simulink model "BlocoHidraulicoLAC_closeLoop"  (R2026a)
settings: Solver=ode15s  StopTime=5  FixedStep=0.001  MaxStep=1e-4
values from neighbouring files (symbols this model uses):
  Gamma = sys_d.B    [sintese_lqi_luenberger_lac.m]    (also in sintese_lqi_luenberger_lac_bateria_de_ensaio.m)
  K_i = -K_aug(3)    [sintese_lqi_luenberger_lac.m]    (also in sintese_lqi_luenberger_lac_bateria_de_ensaio.m)
  K_lqr = [K_pos, K_vel]    [sintese_lqi_luenberger_lac.m]    (also in sintese_lqi_luenberger_lac_bateria_de_ensaio.m)
  L_obs = place(Phi', Cx', polos_obs)'    [sintese_lqi_luenberger_lac.m]    (also in sintese_lqi_luenberger_lac_bateria_de_ensaio.m)
  Phi = sys_d.A    [sintese_lqi_luenberger_lac.m]    (also in sintese_lqi_luenberger_lac_bateria_de_ensaio.m)
undefined symbols (not defined in the file or in its folder): sigbuilder_block
(part 4 of 4)

== matlab function BlocoHidraulicoLAC_closeLoop/ BlocoHidraulicoLAC 2 ==
  settings: updateMethod=DISCRETE
  data: duty_cycle_lac input; u_mcv input; u_pfv input; u_irl input; u_orl input; P_supply output; P_roda output; dt input; x_mm output
function [ P_supply, P_roda, x_mm] = fcn(duty_cycle_lac,u_mcv, u_pfv, u_irl, u_orl,  dt)
%#codegen
% BLOCO DE PLANTA FÍSICA HIDRO-MECÂNICA ATUALIZADO (CINEMÁTICA DO FUSO REAL)
% Inputs:
%   u_mcv, u_pfv, u_irl, u_orl : Sinais ON/OFF (0 ou 1)
%   duty_cycle_lac             : Sinal de comando do LAC (-1.0 a 1.0 ou 0 a 1)
%   dt                         : Passo de amostragem (ex: 0.001)
% Outputs:
%   x_ponto                    : Velocidade instantânea do êmbolo [m/s]
%   P_supply                   : Pressão de suprimento (Nó p1) [Pa]
%   P_roda                     : Pressão na roda (Nó p3) [Pa]
%   x_mm                       : DESLOCAMENTO DO LAC EM MILÍMETROS [mm]

%% 1. PARAMETROS FIXOS DO SISTEMA (Valores validados pelo usuário)
rho     = 850;          % Densidade do fluido [kg/m^3]
beta    = 1.5e9;        % Módulo volumétrico [Pa]
A_lac   = 2.85e-4;      % Área do êmbolo do LAC [m^2]
V10     = 2.0e-5;       % Volume morto inicial [m^3]
%Valor sugerido para teste: Mude de V10 = 2.0e-5 para V10 = 1.0e-5 (\(10\text{ mL}\)).

% % Parâmetro Mecânico Real do Motor/Fuso
% K_drv   = 0.7e-4;      % Ganho real: m/s por unidade de comando (Velocidade máx: 0.269 mm/s)
% tau_m   = 0.020;        % Constante de tempo elétrica/mecânica do motor (ex: 20 ms)

% Parâmetros Reais Extraídos da Bancada (Escala 0-100)
K_drv   = 0.085;    % Média calibrada para a zona útil de controle (10% a 30%)
tau_m   = 0.140;      % Constante de aceleração real do motor (140 ms)

% Válvulas (Orifícios)
Cd      = 0.62;         %1.0;          % Coeficiente de descarga uniforme
A_max   = 3.5e-6;      %8.47e-7;      % Área máxima de passagem das válvulas [m^2]
tau_v   = 0.005;        % Constante de tempo do carretel [s]
pr      = 0.0;          % Pressão do reservatório [Pa]

% Volumes e Compliances dos Nós 2 e 3
C2      = 5.0e-12;      % Compliance da linha principal [m^3/Pa]
% C2      = 2.0e-12;      % REDUZIDO: Linha principal do bloco mais rígida
C3      = 4.5e-12; %2.5e-11;      % Compliance total do caliper [m^3/Pa]
% Valor sugerido para teste: Experimente testar C3 = 1.2e-12 ou C3 = 8.5e-13.


%% 2. INICIALIZAÇÃO DOS ESTADOS INTERNOS (PERSISTENT)
persistent p1 p2 p3 x x_dot a_mcv a_pfv a_irl a_orl

if isempty(p1)
    p1     = 0.0;  p2    = 0.0;  p3    = 0.0;
    x      = 0.0;  x_dot = 0.0;
    a_mcv  = 0.0;  a_pfv = 0.0;  a_irl = 0.0;  a_orl = 0.0;
end

%% 3. DINÂMICA DOS CARRETÉIS DAS VÁLVULAS
a_mcv = a_mcv + (dt / tau_v) * (-a_mcv + double(u_mcv));
a_pfv = a_pfv + (dt / tau_v) * (-a_pfv + double(u_pfv));
a_irl = a_irl + (dt / tau_v) * (-a_irl + double(u_irl));
a_orl = a_orl + (dt / tau_v) * (-a_orl + double(u_orl));

a_mcv = max(0.0, min(1.0, a_mcv));
a_pfv = max(0.0, min(1.0, a_pfv));
a_irl = max(0.0, min(1.0, a_irl));
a_orl = max(0.0, min(1.0, a_orl));

%% 4. CÁLCULO DAS VAZÕES INSTANTÂNEAS
A_eff_mcv = a_mcv * A_max;
A_eff_pfv = a_pfv * A_max;
A_eff_irl = a_irl * A_max; % Acoplamento IRL/ORL conforme lógica
A_eff_orl = a_orl * A_max;

dp_pfv = p1 - p2;
dp_mcv = p2 - pr;
dp_irl = p2 - p3;
dp_orl = p3 - pr;

Q_pfv = Cd * A_eff_pfv * sign(dp_pfv) * sqrt(2 * abs(dp_pfv) / rho);
Q_mcv = Cd * A_eff_mcv * sign(dp_mcv) * sqrt(2 * abs(dp_mcv) / rho);
Q_irl = Cd * A_eff_irl * sign(dp_irl) * sqrt(2 * abs(dp_irl) / rho);
Q_orl = Cd * A_eff_orl * sign(dp_orl) * sqrt(2 * abs(dp_orl) / rho);

%% 5. EQUAÇÕES DIFERENCIAIS DA PLANTA (EDOs)

% --- Mecânica Cinemática Real do Atuador do LAC ---
% Em vez de força, o comando de PWM gera uma velocidade alvo ditada pelo fuso.
% O motor possui um pequeno atraso físico de resposta (atraso de primeira ordem tau_m)
%x_dot_alvo = double(duty_cycle_lac) * K_drv;
x_dot_alvo = (double(duty_cycle_lac) / 100) * K_drv; % Garante que 50 vire 0.5

x_ddot     = (1 / tau_m) * (-x_dot + x_dot_alvo);

% --- Dinâmica Hidráulica ---
V1 = V10 - A_lac * x;
if V1 < 1.0e-7
    V1 = 1.0e-7;
end
p1_dot = (beta / V1) * (A_lac * x_dot - Q_pfv);
p2_dot = (1 / C2) * (Q_pfv - Q_mcv - Q_irl);
p3_dot = (1 / C3) * (Q_irl - Q_orl);

%% 6. INTEGRAÇÃO NUMÉRICA (Método de Euler)
x_dot = x_dot + x_ddot * dt;
x     = x + x_dot * dt;

% [ADICIONE ESTA LINHA AQUI]: Proteção de Fim de Curso Máximo do LAC
if x >= 0.0537
    x = 0.0537;
    x_dot = max(0.0, x_dot); % Impede o pistão de continuar avançando se bater no fundo
end

p1    = p1 + p1_dot * dt;
p2    = p2 + p2_dot * dt;
p3    = p3 + p3_dot * dt;

% Saturações físicas de fim de curso e cavitação
p1 = max(0.0, p1);
p2 = max(0.0, p2);
p3 = max(0.0, p3);
x  = max(0.0, x); % Impede deslocamento negativo na parede inicial

%% 7. ATRIBUIÇÃO DAS SAÍDAS DO BLOCO
%x_ponto  = x_dot;
P_supply = p1/6894.757;
P_roda   = p3/6894.757;
x_mm     = x * 1000; % Converte de metros [m] para milímetros [mm] para leitura real

end



% esse codigo funcionou parcialmente
% function [P_supply, P_roda, x_ponto] = fcn(duty_cycle_lac, u_mcv, u_pfv, u_irl, u_orl,  dt)
% %#codegen
% % BLOCO DE PLANTA FÍSICA HIDRO-MECÂNICA (LAC + VALVULAS + CALIPER)
% % Inputs vindos da ECU:
% %   u_mcv, u_pfv, u_irl, u_orl : Sinais ON/OFF (0 ou 1)
% %   duty_cycle_lac             : Sinal PWM do motor do LAC (0.0 a 1.0)
% %   dt                         : Passo de amostragem da simulação (ex: 0.001)
% % Outputs para os sensores:
% %   x_ponto                    : Velocidade do êmbolo do LAC [m/s]
% %   P_supply                   : Pressão de suprimento (Nó p1 do LAC) [Pa]
% %   P_roda                     : Pressão na roda/caliper (Nó p3) [Pa]
% 
% %% 1. PARAMETROS FIXOS DO SISTEMA (Altere conforme seu projeto)
% % Fluido e Geometria do LAC
% rho     = 850;          % Densidade do fluido [kg/m^3]
% beta    = 1.5e9;        % Módulo volumétrico [Pa]
% A_lac   = 2.85e-4;       % Área do êmbolo do LAC [m^2]
% V10     = 2.0e-5;       % Volume morto inicial [m^3]
% 
% % Mecânica do Atuador do LAC
% m_lac   = 1.5;          % Massa equivalente do êmbolo/motor [kg]
% b_lac   = 2000;          % Coeficiente de amortecimento [N*s/m]
% k_lac   = 0.0;          % Rigidez de retorno mecânico [N/m]
% K_motor = 0.538;          % Ganho de força do motor por Duty Cycle [N]
% V_max   = 24;           % Tensão de alimentação nominal [V]
% 
% % Válvulas (Orifícios)
% Cd      = 1.0;         % Coeficiente de descarga uniforme
% A_max   = 8.47e-7;      % Área máxima de passagem das válvulas [m^2]
% tau_v   = 0.005;        % Constante de tempo do carretel [s]
% pr      = 0.0;          % Pressão do reservatório [Pa]
% 
% % Volumes e Compliances dos Nós 2 e 3
% C2      = 5.0e-12;      % Compliance da linha principal [m^3/Pa]
% C3      = 2.5e-11;      % Compliance total do caliper (Fluido + Pastilha) [m^3/Pa]
% 
% %% 2. INICIALIZAÇÃO DOS ESTADOS INTERNOS (PERSISTENT)
% persistent p1 p2 p3 x x_dot a_mcv a_pfv a_irl a_orl
% 
% if isempty(p1)
%     p1     = 0.0;  p2    = 0.0;  p3    = 0.0;
%     x      = 0.0;  x_dot = 0.0;
%     a_mcv  = 0.0;  a_pfv = 0.0;  a_irl = 0.0;  a_orl = 0.0;
% end
% 
% %% 3. DINÂMICA DOS CARRETÉIS DAS VÁLVULAS (Filtros de comando)
% a_mcv = a_mcv + (dt / tau_v) * (-a_mcv + double(u_mcv));
% a_pfv = a_pfv + (dt / tau_v) * (-a_pfv + double(u_pfv));
% a_irl = a_irl + (dt / tau_v) * (-a_irl + double(u_irl));
% a_orl = a_orl + (dt / tau_v) * (-a_orl + double(u_orl));
% 
% % Garantir limites físicos das aberturas [0, 1]
% a_mcv = max(0.0, min(1.0, a_mcv));
% a_pfv = max(0.0, min(1.0, a_pfv));
% a_irl = max(0.0, min(1.0, a_irl));
% a_orl = max(0.0, min(1.0, a_orl));
% 
% %% 4. CÁLCULO DAS VAZÕES INSTANTÂNEAS (Modelo de Orifício)
% % Áreas instantâneas
% A_eff_mcv = a_mcv * A_max;
% A_eff_pfv = a_pfv * A_max;
% A_eff_irl = a_irl * A_max;
% A_eff_orl = a_orl * A_max;
% 
% % Diferenciais de pressão
% dp_pfv = p1 - p2;
% dp_mcv = p2 - pr;
% dp_irl = p2 - p3;
% dp_orl = p3 - pr;
% 
% % Equação de escoamento não-linear
% Q_pfv = Cd * A_eff_pfv * sign(dp_pfv) * sqrt(2 * abs(dp_pfv) / rho);
% Q_mcv = Cd * A_eff_mcv * sign(dp_mcv) * sqrt(2 * abs(dp_mcv) / rho);
% Q_irl = Cd * A_eff_irl * sign(dp_irl) * sqrt(2 * abs(dp_irl) / rho);
% Q_orl = Cd * A_eff_orl * sign(dp_orl) * sqrt(2 * abs(dp_orl) / rho);
% 
% %% 5. EQUAÇÕES DIFERENCIAIS DA PLANTA (EDOs)
% 
% % --- Dinâmica Mecânica do LAC ---
% % Força elétrica gerada pelo PWM (Limitada entre 0 e K_motor)
% F_motor = double(max(0.0, min(1.0, duty_cycle_lac))) * K_motor;
% % Força de reação hidráulica contrária que o fluido faz no êmbolo
% F_hidr  = A_lac * p1; 
% 
% % Aceleração do LAC (x_ponto_ponto)
% x_ddot = (1 / m_lac) * (F_motor - b_lac * x_dot - k_lac * x - F_hidr);
% 
% % --- Dinâmica Hidráulica (Pressões) ---
% % Nó 1: Volume variável do LAC
% V1 = V10 - A_lac * x;
% if V1 < 1.0e-7 % Proteção contra fim de curso/divisão por zero
%     V1 = 1.0e-7;
% end
% p1_dot = (beta / V1) * (A_lac * x_dot - Q_pfv);
% 
% % Nó 2: Linha principal
% p2_dot = (1 / C2) * (Q_pfv - Q_mcv - Q_irl);
% 
% % Nó 3: Caliper da Roda
% p3_dot = (1 / C3) * (Q_irl - Q_orl);
% 
% %% 6. INTEGRAÇÃO NUMÉRICA (Método de Euler)
% x_dot = x_dot + x_ddot * dt;
% x     = x + x_dot * dt;
% p1    = p1 + p1_dot * dt;
% p2    = p2 + p2_dot * dt;
% p3    = p3 + p3_dot * dt;
% 
% % Saturações de segurança física (Pressão não pode ser negativa -> Cavitação)
% p1 = max(0.0, p1);
% p2 = max(0.0, p2);
% p3 = max(0.0, p3);
% x  = max(0.0, x); % Êmbolo não volta além da posição de repouso
% 
% %% 7. ATRIBUIÇÃO DAS SAÍDAS DO BLOCO
% x_ponto  = x_dot;
% P_supply = p1/6894.757;
% P_roda   = p3/6894.757;
% 
% end










% function [Pw_psi, Ps_psi, x_mm] = MKc2_step(PWM, MCV, PFV, IRL, ORL)
% %#codegen
% % Planta hidráulica de freio (AEB/ACC) simplificada: LAC + válvulas + caliper
% % Entradas:
% %   PWM ∈ [0..100] ou [0..1]  (comando do LAC)
% %   MCV, PFV, IRL, ORL ∈ {0,1} (1=acionada)
% % Convenção:
% %   MCV=1 isola do reservatório (sem alívio); MCV=0 abre LAC→reservatório
% %   PFV=1 abre LAC→linha; IRL=1 abre linha→caliper; ORL=1 abre caliper→reservatório
% % Saídas:
% %   Pw_psi (psi) — pressão na roda/caliper
% %   Ps_psi (psi) — pressão de suprimento (câmara do LAC)
% %   x_mm   (mm)  — deslocamento do LAC
% 
% % ---------------------------------
% % ESTADOS
% % ---------------------------------
% persistent x Ps Pw Vgap a_line a_orl a_mcv
% if isempty(x)
%     x     = 0.0;    % m
%     Ps    = 0.0;    % Pa
%     Pw    = 0.0;    % Pa
%     Vgap  = 6.3e-6; % m^3 (≈ 6.3 mL) — folga inicial da roda (ajuste)
%     a_line= 0.0;    % m^2 área efetiva S↔W (PFV∧IRL)
%     a_orl = 0.0;    % m^2 área efetiva W→R (ORL)
%     a_mcv = 0.0;    % m^2 área efetiva S→R (MCV aberta)
% end
% 
% % ---------------------------------
% % PARÂMETROS (ajuste para o hardware)
% % ---------------------------------
% % Discretização
% Ts = 1e-3;                  % s
% 
% % LAC (cinemática aberta, sem PI interno)
% A_p   = 2.85e-4;            % m^2 (área efetiva do pistão)
% x_max = 0.0537;             % m  (curso máx)
% x_ds  = 0.0050;             % m  (dead stroke visto no LAC)
% K_drv_mps_per_pct = 2.69e-4;% m/s por %PWM (caracterizado no real)
% F_max = 2500.0;             % N  (força máx no êmbolo a 100% PWM) — ajuste
% use_droop = true;           % queda de velocidade com pressão (v→0 quando A_p*Ps→F_max)
% 
% % Fluido / compressibilidade efetiva
% rho     = 1050.0;           % kg/m^3
% betaS0  = 1.0e9;            % Pa    (suprimento)
% betaW0  = 1.0e9;            % Pa    (roda)
% k_betaS = 0.0e-9;           % 1/Pa  (enrijecimento com P) — ajuste fino
% k_betaW = 2.0e-9;           % 1/Pa  (enrijecimento com P) — ajuste fino
% Vs0     = 4.0e-6;           % m^3   (volume efetivo suprimento)
% Vw0     = 11.3e-6;          % m^3   (volume efetivo roda/linha, sem folga)
% 
% % Orifícios equivalentes (Cd*A) em ON (65 cm^3/s @ 25 bar → ~9.4e-7 m^2)
% CdA_LINE_ON = 9.4e-7;       % m^2 (S↔W quando PFV∧IRL abertos)
% CdA_ORL_ON  = 9.4e-7;       % m^2 (W→R quando ORL aberta)
% CdA_MCV_ON  = 9.4e-7;       % m^2 (S→R quando MCV aberta)
% 
% % Fugas (opcionais)
% CdA_leak_S  = 0.0e-9;       % m^2 (S→R)
% CdA_leak_W  = 0.0e-9;       % m^2 (W→R)
% 
% % Dinâmica eletromecânica das válvulas (1ª ordem)
% tau_val = 0.02;             % s (10–30 ms típico)
% 
% % Conversão
% PA_PER_PSI = 6894.757;
% 
% % ---------------------------------
% % ENTRADAS E FLAGS
% % ---------------------------------
% % PWM como %
% if PWM <= 1.0
%     pwm_pct = 100.0*max(0.0,min(1.0,PWM));
% else
%     pwm_pct = max(0.0,min(100.0,PWM));
% end
% 
% MCV_isol = (MCV ~= 0);  % 1=isola
% PFV_open = (PFV ~= 0);  % 1=aberta
% IRL_open = (IRL ~= 0);  % 1=aberta
% ORL_open = (ORL ~= 0);  % 1=aberta
% 
% % ---------------------------------
% % LAC — deslocamento a partir do PWM (com droop de carga)
% % ---------------------------------
% P_port = Ps;           % pressão na face do êmbolo (≈Ps se MCV=1; ≈0 se MCV=0)
% if ~MCV_isol
%     P_port = 0.0;
% end
% 
% v_nom = K_drv_mps_per_pct * pwm_pct;   % m/s
% if use_droop
%     droop = max(0.0, 1.0 - (A_p*P_port)/max(F_max,1.0));
% else
%     droop = 1.0;
% end
% v = v_nom * droop;                     % m/s
% 
% % integrar x com saturação
% x = x + Ts*v;
% if x < 0.0,    x = 0.0;    end
% if x > x_max,  x = x_max;  end
% 
% % Vazão do pistão (só após dead stroke)
% if x <= x_ds
%     Qp = 0.0;
% else
%     Qp = A_p * v;   % m^3/s
% end
% 
% % ---------------------------------
% % Válvulas — áreas efetivas com atraso (1ª ordem)
% % ---------------------------------
% line_cmd = CdA_LINE_ON * double(PFV_open && IRL_open);
% orl_cmd  = CdA_ORL_ON  * double(ORL_open);
% mcv_cmd  = CdA_MCV_ON  * double(~MCV_isol);
% 
% a_line = a_line + Ts*(line_cmd - a_line)/max(tau_val,Ts);
% a_orl  = a_orl  + Ts*(orl_cmd  - a_orl )/max(tau_val,Ts);
% a_mcv  = a_mcv  + Ts*(mcv_cmd  - a_mcv )/max(tau_val,Ts);
% 
% % ---------------------------------
% % Lei de orifício — vazões assinadas
% % ---------------------------------
% % Enquanto houver folga (Vgap>0), a pressão na roda é ~0.
% Pw_for_line = Pw;
% if Vgap > 0.0
%     Pw_for_line = 0.0;
% end
% 
% Q_sw   = orifice_signed(Ps, Pw_for_line, a_line, rho);  % S↔W
% Q_wr   = orifice_signed(Pw, 0.0,       a_orl,  rho);    % W→R
% Q_sr   = orifice_signed(Ps, 0.0,       a_mcv,  rho);    % S→R
% Q_lk_S = orifice_signed(Ps, 0.0,       CdA_leak_S, rho);
% Q_lk_W = orifice_signed(Pw, 0.0,       CdA_leak_W, rho);
% 
% % ---------------------------------
% % Dead stroke como volume de folga (consome Q_sw até zerar Vgap)
% % ---------------------------------
% if (Vgap > 0.0) && (Q_sw > 0.0) && (a_line > 0.0)
%     Vgap = Vgap - Ts*Q_sw;
%     if Vgap < 0.0, Vgap = 0.0; end
% end
% 
% % ---------------------------------
% % Balanço de compressibilidade
% % ---------------------------------
% betaS = betaS0 * (1.0 + k_betaS*Ps);
% betaW = betaW0 * (1.0 + k_betaW*Pw);
% 
% % Suprimento (sempre integra)
% Ps_dot = (betaS / max(Vs0,eps)) * ( Qp - Q_sr - Q_sw - Q_lk_S );
% Ps = Ps + Ts*Ps_dot;
% if Ps < 0.0, Ps = 0.0; end
% 
% % Roda: só integra após fechar folga; antes, mantém Pw≈0
% if Vgap > 0.0
%     Pw = 0.0;
% else
%     Pw_dot = (betaW / max(Vw0,eps)) * ( Q_sw - Q_wr - Q_lk_W );
%     Pw = Pw + Ts*Pw_dot;
%     if Pw < 0.0, Pw = 0.0; end
% end
% 
% % ---------------------------------
% % SAÍDAS
% % ---------------------------------
% Pw_psi = Pw / PA_PER_PSI;
% Ps_psi = Ps / PA_PER_PSI;
% x_mm   = x  * 1e3;
% 
% end
% 
% % -------- orifício com sinal (local) --------
% function q = orifice_signed(Pu, Pd, CdA, rho)
% %#codegen
% if CdA <= 0.0
%     q = 0.0;
%     return;
% end
% dP = Pu - Pd;
% if dP > 0.0
%     q = CdA * sqrt(2.0 * dP / rho);
% elseif dP < 0.0
%     q = -CdA * sqrt(2.0 * (-dP) / rho);
% else
%     q = 0.0;
% end
% end
% % function [Pw_psi, Ps_psi, x_mm] = MKc2_step(PWM, MCV, PFV, IRL, ORL)
% % %#codegen
% % % Planta hidráulica MKc2 (LAC + válvulas) sem controle, com lei de orifício.
% % % Entradas (escalares):
% % %   PWM ∈ [0..100] (%) ou [0..1]       – comando do motor do LAC (abrevia: velocidade)
% % %   MCV, PFV, IRL, ORL ∈ {0,1}         – válvulas ON/OFF (1=acionada)
% % % Convenção das válvulas (compatível com o prompt):
% % %   MCV: 1=isola reservatório (câmara do LAC fechada); 0=alívio LAC→reservatório
% % %   PFV: 1=abre LAC→linha
% % %   IRL: 1=abre linha→caliper (convenção pedida: 1=ABERTA)
% % %   ORL: 1=abre caliper→reservatório
% % % Saídas:
% % %   Pw_psi – pressão no caliper (psi)
% % %   Ps_psi – pressão de suprimento/câmara do LAC (psi)
% % %   x_mm   – deslocamento do LAC (mm)
% % 
% % % ==========================
% % % ESTADOS (persistentes)
% % % ==========================
% % persistent x Ps Pw
% % if isempty(x)
% %     x  = 0.0;   % m  (posição do LAC)
% %     Ps = 0.0;   % Pa (pressão na câmara do LAC / suprimento)
% %     Pw = 0.0;   % Pa (pressão na roda/caliper)
% % end
% % 
% % % ==========================
% % % PARÂMETROS (ajustáveis)
% % % ==========================
% % % Discretização
% % Ts = 1e-3;                  % s (use igual ao passo do modelo)
% % 
% % % LAC (geometria e curso)
% % A_p   = 2.85e-4;            % m^2  (área efetiva do pistão do LAC)
% % x_max = 0.0537;             % m    (curso máximo ~53,7 mm)
% % x_ds  = 0.0050;             % m    (dead stroke ~5,0 mm – sem geração de pressão)
% % 
% % % LAC (cinemática aberta – sem PI dentro do bloco)
% % % K_drv dado em m/s por %PWM (valores coletados do sistema)
% % K_drv_mps_per_pct = 2.69e-4;   % m/s por %PWM
% % 
% % % Fluido / compressibilidade efetiva (ajuste pela validação)
% % rho   = 1050.0;             % kg/m^3
% % betaS = 1.0e9;              % Pa (módulo efetivo nó S – LAC)
% % betaW = 1.0e9;              % Pa (módulo efetivo nó W – roda)
% % Vs0   = 4.0e-6;             % m^3 (volume efetivo no nó S – ordem de mL)
% % Vw0   = 11.3e-6;            % m^3 (volume efetivo no nó W – ~ V_line_dead + V_dead_max)
% % 
% % % Orifícios equivalentes (Cd*A) quando ABERTOS (valores a partir de 65 cm^3/s @ 25 bar)
% % % CdA ≈ Q_nom / sqrt(2*ΔP/ρ) → ≈ 9.4e-7 m^2 (ajuste fino em bancada/simulação)
% % CdA_LINE_ON = 9.4e-7;       % m^2 (PFV & IRL ABERTAS: LAC ↔ caliper)
% % CdA_ORL_ON  = 9.4e-7;       % m^2 (ORL ABERTA: caliper → reservatório)
% % CdA_MCV_ON  = 9.4e-7;       % m^2 (MCV ABERTA: LAC → reservatório)
% % 
% % % Fugas pequenas (opcionais; ajudam estabilidade numérica)
% % CdA_leak_S  = 0.0e-9;       % m^2 (fuga S→reservatório)
% % CdA_leak_W  = 0.0e-9;       % m^2 (fuga W→reservatório)
% % 
% % % Conversão
% % PA_PER_PSI = 6894.757;      % Pa/psi
% % 
% % % ==========================
% % % PROCESSAMENTO DE ENTRADAS
% % % ==========================
% % % Normalização de PWM (aceita % ou [0..1])
% % if PWM > 1.0
% %     pwm_pct = PWM;           % já está em %
% % else
% %     pwm_pct = 100.0*PWM;     % converte fração → %
% % end
% % if pwm_pct < 0.0;   pwm_pct = 0.0;   end
% % if pwm_pct > 100.0; pwm_pct = 100.0; end
% % 
% % % Flags de válvula (1=ON)
% % MCV_isol = (MCV ~= 0);   % 1=isola (fechada p/ reservatório)
% % PFV_open = (PFV ~= 0);   % 1=aberta
% % IRL_open = (IRL ~= 0);   % 1=aberta (convenção pedida)
% % ORL_open = (ORL ~= 0);   % 1=aberta
% % 
% % % ==========================
% % % CINEMÁTICA DO LAC (sem PI)
% % % ==========================
% % % Fonte de velocidade: v = K_drv * (%PWM)
% % v_cmd = K_drv_mps_per_pct * pwm_pct;   % m/s (sempre positiva neste modelo)
% % 
% % % Integração de posição com saturação mecânica
% % x = x + Ts * v_cmd;
% % if x < 0.0
% %     x = 0.0;
% % end
% % if x > x_max
% %     x = x_max;
% % end
% % 
% % % Vazão volumétrica do pistão (só após dead stroke)
% % if x <= x_ds
% %     Qp = 0.0;            % m^3/s – tomando folgas; sem geração de pressão
% % else
% %     Qp = A_p * v_cmd;    % m^3/s – fluxo injetado no nó S
% % end
% % 
% % % ==========================
% % % HIDRÁULICA – LEI DE ORIFÍCIO
% % % ==========================
% % % Áreas ativas conforme comandos
% % CdA_line = 0.0;
% % if PFV_open && IRL_open
% %     CdA_line = CdA_LINE_ON;      % LAC ↔ roda
% % end
% % 
% % CdA_orl = 0.0;
% % if ORL_open
% %     CdA_orl = CdA_ORL_ON;        % roda → reservatório
% % end
% % 
% % CdA_mcv = 0.0;
% % if ~MCV_isol
% %     CdA_mcv = CdA_MCV_ON;        % LAC → reservatório
% % end
% % 
% % % Vazões assinadas (sentido positivo do primeiro nó para o segundo)
% % % Nodos: S (Ps), W (Pw), R (Pr≈0)
% % Pr  = 0.0;
% % Q_sw = orifice_signed(Ps, Pw, CdA_line, rho);   % S→W
% % Q_wr = orifice_signed(Pw, Pr,  CdA_orl,  rho);  % W→R
% % Q_sr = orifice_signed(Ps, Pr,  CdA_mcv,  rho);  % S→R
% % 
% % % Fugas (sempre para reservatório)
% % Q_leak_S = orifice_signed(Ps, Pr, CdA_leak_S, rho);
% % Q_leak_W = orifice_signed(Pw, Pr, CdA_leak_W, rho);
% % 
% % % Balanço de massa/compressibilidade
% % % dP/dt = (β/V) * (ΣQ_entrada − ΣQ_saída)
% % Ps_dot = (betaS / Vs0) * ( Qp - Q_sr - Q_sw - Q_leak_S );
% % Pw_dot = (betaW / Vw0) * ( Q_sw - Q_wr - Q_leak_W );
% % 
% % % Integração de pressões
% % Ps = Ps + Ts * Ps_dot;
% % Pw = Pw + Ts * Pw_dot;
% % 
% % % Limites físicos
% % if Ps < 0.0; Ps = 0.0; end
% % if Pw < 0.0; Pw = 0.0; end
% % 
% % % ==========================
% % % SAÍDAS
% % % ==========================
% % Pw_psi = Pw / PA_PER_PSI;
% % Ps_psi = Ps / PA_PER_PSI;
% % x_mm   = x  * 1e3;
% % 
% % 
% % 
% % 
% % 
% % 
% % 
% % 
% % 
% % 
% % 
% % 
% % 
% % 
% % 
% % 
% % 
% % 
% % 
% % 
% % 
% % Ps_dot = (Ps_beta_s/Vs) * ( Qp - Q_sr - sum_i * Q_swi - Q_leak_S );
% % Pwi_dot = (Pwi_beta_w_i/Vw_i) * ( Q_swi - Q_wri - Q_leak_Wi );
% % 
% % 
% % end
% % 
% % % ==========================
% % % Função local: lei de orifício com sinal
% % % q > 0 quando Pu>Pd (escoa de Pu→Pd); q < 0 quando Pu<Pd.
% % % ==========================
% % function q = orifice_signed(Pu, Pd, CdA, rho)
% % %#codegen
% % if CdA <= 0.0
% %     q = 0.0;
% %     return;
% % end
% % dP = Pu - Pd;
% % if dP > 0.0
% %     q = CdA * sqrt(2.0 * dP / rho);
% % elseif dP < 0.0
% %     q = -CdA * sqrt(2.0 * (-dP) / rho);
% % else
% %     q = 0.0;
% % end
% % end
% % 
% % % function [Pw_psi, Ps_psi, x_mm] = MKc2_step(PWM, MCV, PFV, IRL, ORL)
% % % %#codegen
% % % % MKc2_step — planta hidráulica (LAC + válvulas) com lei de orifício, pronta p/ portabilidade
% % % % Entradas (escalares):
% % % %   PWM ∈ [0..100] (%) ou [0..1]   — comando do motor/atuador do LAC
% % % %   MCV, PFV, IRL, ORL ∈ {0,1}     — comandos ON/OFF das válvulas
% % % % Saídas:
% % % %   Pw_psi — pressão no caliper (psi)
% % % %   Ps_psi — pressão na câmara do LAC (psi)
% % % %   x_mm   — deslocamento do LAC (mm)
% % % 
% % % % ESTADOS
% % % persistent x v Ps Pw
% % % if isempty(x)
% % %     x  = 0.0;   % m
% % %     v  = 0.0;   % m/s
% % %     Ps = 0.0;   % Pa
% % %     Pw = 0.0;   % Pa
% % % end
% % % 
% % % % ==========================
% % % % PARÂMETROS AJUSTÁVEIS
% % % % ==========================
% % % % Discretização
% % % Ts = 1e-3;        % s (use o mesmo passo do modelo)
% % % 
% % % % Mecânica do LAC
% % % x_max = 0.043;    % m (curso máximo 43 mm)
% % % x_ds  = 0.005;    % m (dead stroke 5 mm)
% % % M_eq  = 0.50;     % kg (massa/inerção equivalente)
% % % B_m   = 20.0;     % N*s/m (atrito viscoso)
% % % K_f   = 200.0;    % N (força efetiva do atuador a PWM=1)
% % % A_p   = 1.0e-4;   % m^2 (área efetiva do êmbolo ~ diâmetro ≈ 11.3 mm)
% % % 
% % % % Hidráulica (compressibilidade e volumes efetivos)
% % % beta_s = 1.5e9;   % Pa (módulo volumétrico efetivo da câmara do LAC)
% % % beta_w = 1.5e9;   % Pa (módulo volumétrico efetivo do caliper/linha roda)
% % % Vs0    = 4.0e-6;  % m^3 (volume efetivo câmara LAC ~ 4 mL)
% % % Vw0    = 12.0e-6; % m^3 (volume efetivo caliper/linha ~ 12 mL)
% % % rho    = 1050.0;  % kg/m^3 (densidade do fluido)
% % % Pr     = 0.0;     % Pa (reservatório em pressão de referência ≈ 0 gauge)
% % % 
% % % % Áreas efetivas de orifício (Cd*A) quando ABERTAS (ON):
% % % CdA_LINE_ON = 1.0e-7;  % m^2 (linha LAC↔caliper, PFV e IRL ABERTAS)
% % % CdA_ORL_ON  = 1.2e-7;  % m^2 (retorno caliper→reservatório, ORL ABERTA)
% % % CdA_MCV_ON  = 1.0e-7;  % m^2 (alívio LAC→reservatório, MCV ABERTA)
% % % 
% % % % Pequenas fugas opcionais (mantêm numérica estável quando tudo fechado)
% % % CdA_leak_S  = 0.0e-9;  % m^2 (fuga câmara LAC→reservatório)
% % % CdA_leak_W  = 0.0e-9;  % m^2 (fuga caliper→reservatório)
% % % 
% % % % Conversão
% % % PA_PER_PSI = 6894.757; % Pa/psi
% % % 
% % % % ==========================
% % % % CONVENÇÃO DE COMANDO (PORTABILIDADE)
% % % % 1 = acionado (ON), 0 = desacionado (OFF)
% % % % - MCV=1: isola do reservatório (sem alívio). MCV=0: alívio LAC→reservatório.
% % % % - PFV=1: abre LAC→linha.
% % % % - IRL=1: ABRE para o caliper (convenção pedida). IRL=0: isola caliper.
% % % % - ORL=1: abre retorno caliper→reservatório.
% % % % ==========================
% % % MCV_isol  = (MCV ~= 0);   % MCV=1 isola; MCV=0 alivia
% % % PFV_open  = (PFV ~= 0);   % PFV=1 abre
% % % IRL_open  = (IRL ~= 0);   % IRL=1 abre (conforme solicitado)
% % % ORL_open  = (ORL ~= 0);   % ORL=1 abre
% % % 
% % % % Normalização PWM
% % % if PWM > 1.0
% % %     PWM = PWM/100.0;
% % % end
% % % if PWM < 0.0; PWM = 0.0; end
% % % if PWM > 1.0; PWM = 1.0; end
% % % 
% % % % ==========================
% % % % MECÂNICA DO LAC
% % % % ==========================
% % % % Reação hidráulica no êmbolo (porto da câmara do LAC)
% % % P_port = Ps;
% % % 
% % % % Forças e aceleração
% % % F_m = K_f * PWM;              % N (atuador)
% % % F_h = A_p * P_port;           % N (reação do fluido)
% % % a   = (F_m - B_m*v - F_h)/M_eq;
% % % 
% % % % Integração com saturações de curso
% % % v = v + Ts*a;
% % % x = x + Ts*v;
% % % 
% % % if x < 0.0
% % %     x = 0.0;
% % %     if v < 0.0; v = 0.0; end
% % % end
% % % if x > x_max
% % %     x = x_max;
% % %     if v > 0.0; v = 0.0; end
% % % end
% % % 
% % % % Vazão do êmbolo (só conta após dead stroke)
% % % if x <= x_ds
% % %     Qp = 0.0;      % m^3/s (tomada de folgas; não gera pressão)
% % % else
% % %     Qp = A_p * v;  % m^3/s (assinada: positiva comprime, negativa suga)
% % % end
% % % 
% % % % ==========================
% % % % HIDRÁULICA COM LEI DE ORIFÍCIO
% % % % ==========================
% % % % Áreas ativas conforme comandos
% % % CdA_line = 0.0;
% % % if PFV_open && IRL_open
% % %     CdA_line = CdA_LINE_ON;
% % % end
% % % 
% % % CdA_orl = 0.0;
% % % if ORL_open
% % %     CdA_orl = CdA_ORL_ON;
% % % end
% % % 
% % % CdA_mcv = 0.0;
% % % if ~MCV_isol
% % %     % MCV aberta ao reservatório ⇒ alívio LAC→reservatório
% % %     CdA_mcv = CdA_MCV_ON;
% % % end
% % % 
% % % % Vazões (assinadas pelo gradiente de pressão)
% % % Q_sw = orifice_signed(Ps, Pw, CdA_line, rho);      % S→W (positivo se Ps>Pw)
% % % Q_wr = orifice_signed(Pw, Pr,  CdA_orl,  rho);     % W→R (positivo se Pw>Pr)
% % % Q_sr = orifice_signed(Ps, Pr,  CdA_mcv,  rho);     % S→R (positivo se Ps>Pr)
% % % 
% % % % Fugas opcionais (sempre para reservatório)
% % % Q_leak_S = orifice_signed(Ps, Pr, CdA_leak_S, rho);
% % % Q_leak_W = orifice_signed(Pw, Pr, CdA_leak_W, rho);
% % % 
% % % % Balanços de volume (compressibilidade)
% % % Ps_dot = (beta_s / Vs0) * ( Qp - Q_sr - Q_sw - Q_leak_S );
% % % Pw_dot = (beta_w / Vw0) * ( Q_sw - Q_wr - Q_leak_W );
% % % 
% % % % Integração de pressões
% % % Ps = Ps + Ts * Ps_dot;
% % % Pw = Pw + Ts * Pw_dot;
% % % 
% % % % Saturações físicas
% % % if Ps < 0.0; Ps = 0.0; end
% % % if Pw < 0.0; Pw = 0.0; end
% % % 
% % % % ==========================
% % % % SAÍDAS
% % % % ==========================
% % % Pw_psi = Pw / PA_PER_PSI;
% % % Ps_psi = Ps / PA_PER_PSI;
% % % x_mm   = x * 1e3;
% % % 
% % % end
% % % 
% % % % ==========================
% % % % Função local: lei de orifício com sinal
% % % %   Retorna vazão positiva no sentido Pu→Pd quando Pu>Pd,
% % % %   e negativa quando Pu<Pd.
% % % % ==========================
% % % function q = orifice_signed(Pu, Pd, CdA, rho)
% % % %#codegen
% % % if CdA <= 0
% % %     q = 0.0;
% % %     return;
% % % end
% % % dP = Pu - Pd;
% % % if dP > 0
% % %     q = CdA * sqrt(2.0 * dP / rho);
% % % elseif dP < 0
% % %     q = -CdA * sqrt(2.0 * (-dP) / rho);
% % % else
% % %     q = 0.0;
% % % end
% % % end
% % % % function [Ps_psi, Pw_psi, x_mm] = MKc2_step(PWM, MCV, PFV, IRL, ORL) 
% % % % % MKc2_step — modelo simplificado (teórico) do módulo hidráulico com LAC e válvulas. 
% % % % % Entradas: 
% % % % % PWM [0..100] (%) ou [0..1], MCV/PFV/IRL/ORL ∈ {0,1} 
% % % % % Saídas: 
% % % % % Pw_psi — pressão no caliper (psi) 
% % % % % Ps_psi — pressão na câmara do LAC (psi) 
% % % % % x_mm — deslocamento do LAC (mm)
% % % % 
% % % % % Estados persistentes 
% % % % persistent x v Ps Pw 
% % % % if isempty(x) 
% % % % 	x = 0.0; % m 
% % % % 	v = 0.0; % m/s 
% % % % 	Ps = 0.0; % Pa 
% % % % 	Pw = 0.0; % Pa 
% % % % end
% % % % 
% % % % % Constantes e parâmetros (ajuste conforme necessário) 
% % % % Ts = 1e-3; % s (usar igual ao sample time do bloco) 
% % % % x_max = 0.043; % m (43 mm) 
% % % % x_ds = 0.005; % m (5 mm dead stroke) 
% % % % M_eq = 0.50; % kg 
% % % % B_m = 20.0; % N*s/m 
% % % % K_f = 200.0; % N (força efetiva max. do atuador no êmbolo) 
% % % % A_p = 1.0e-4; % m^2 (área efetiva do êmbolo) 
% % % % Pmax = 10.3e6; % Pa (~1500 psi) 
% % % % k_p = 250.0; % 1/m (≈0.25 por mm) 
% % % % tau_h = 5e-3; % s (dinâmica hidráulica do LAC) 
% % % % tau_mcv = 3e-3; % s (alívio via MCV) 
% % % % tau_line= 2e-3; % s (equalização LAC↔caliper) 
% % % % tau_orl = 8e-3; % s (alívio via ORL) 
% % % % tau_leak= 0.5; % s (retenção/fuga lenta) 
% % % % PA_PER_PSI = 6894.757; % Pa por psi
% % % % 
% % % % % Normalização PWM para [0,1] 
% % % % if PWM > 1.0 
% % % % 	PWM = PWM/100.0; 
% % % % end 
% % % % if PWM < 0.0 
% % % % 	PWM = 0.0; 
% % % % end 
% % % % if PWM > 1.0 
% % % % 	PWM = 1.0; 	
% % % % end
% % % % 
% % % % % 1) Força do atuador e pressão no porto do LAC (para reação hidráulica) 
% % % % % Assumimos lógica de válvulas: 
% % % % % MCV=1 fecha reservatório (isola); MCV=0 abre (alívio). 
% % % % % PFV=1 abre LAC→linha; IRL=0 abre linha→caliper; ORL=1 alívio caliper→reservatório. 
% % % % % Pressão que reage no êmbolo: 
% % % % if MCV==0 
% % % %     P_port = 0.0; % câmara conectada ao reservatório 
% % % % else % MCV=1: câmara pode estar isolada (PFV=0) ou conectada à linha (PFV=1) 
% % % %     if PFV==1 && IRL==0 && ORL==0 % LAC conectado ao caliper (sem alívio) 
% % % %     % aproximamos reação no êmbolo pela pressão do LAC (Ps), 
% % % %     % que tenderá a equalizar com Pw (feito mais abaixo) 
% % % %         P_port = Ps; 
% % % %     elseif PFV==0 % LAC isolado da linha, câmara fechada 
% % % %         P_port = Ps; 
% % % %     else % Outras combinações (ex.: IRL=1 ou ORL=1) → pouca reação efetiva no êmbolo
% % % %         P_port = Ps; 
% % % %     end 
% % % % end
% % % % 
% % % % F_m = K_f * PWM; % N 
% % % % F_h = A_p * P_port; % N (oposição hidráulica) 
% % % % a = (F_m - B_m*v - F_h)/M_eq; % m/s^2
% % % % 
% % % % % Integração mecânica 
% % % % v = v + Ts*a; 
% % % % x = x + Ts*v;
% % % % 
% % % % % Limites mecânicos (batente e não recuar abaixo de 0) 
% % % % if x < 0.0 
% % % %     x = 0.0; 
% % % % 	if v < 0.0; v = 0.0; 
% % % % 	end 
% % % % end 
% % % % if x > x_max 
% % % %     x = x_max; 
% % % % 	if v > 0.0; v = 0.0; 
% % % % 	end 
% % % % end
% % % % 
% % % % % 2) Pressão alvo no LAC por dead stroke + exponencial 
% % % % if x <= x_ds 
% % % % 	Pstat = 0.0; 
% % % % else 
% % % % 	Pstat = Pmax * (1.0 - exp(-k_p * (x - x_ds))); 
% % % % end
% % % % 
% % % % % 3) Dinâmica da pressão na câmara do LAC (Ps) 
% % % % if MCV==1 % Isolado do reservatório → Ps tende a Pstat 
% % % % 	Ps = Ps + Ts*(Pstat - Ps)/tau_h; 
% % % % else % Aberto ao reservatório → Ps tende a 0 
% % % % 	Ps = Ps + Ts*(0.0 - Ps)/tau_mcv; 
% % % % end 
% % % % if Ps < 0.0 
% % % % 	Ps = 0.0; 
% % % % end
% % % % 
% % % % % 4) Dinâmica da pressão no caliper (Pw) 
% % % % if ORL==1 % Alívio direto ao reservatório domina 
% % % % 	Pw = Pw + Ts*(0.0 - Pw)/tau_orl; 
% % % % else % Sem alívio 
% % % % 	if (IRL==0) && (PFV==1) && (MCV==1) % Linha LAC↔caliper conectada e LAC isolado do reservatório 
% % % % 		Pw = Pw + Ts*(Ps - Pw)/tau_line; 
% % % % 	else % Isolado/retido (IRL=1 ou PFV=0 ou MCV=0) → retenção com fuga lenta 
% % % % 		Pw = Pw + Ts*(0.0 - Pw)/tau_leak; 
% % % % 	end 
% % % % end 
% % % % if Pw < 0.0 
% % % % 	Pw = 0.0; 
% % % % end
% % % % 
% % % % % 5) Saídas convertidas 
% % % % Pw_psi = Pw / PA_PER_PSI; 
% % % % Ps_psi = Ps / PA_PER_PSI; 
% % % % x_mm = x * 1e3;
% % % % 
% % % % end
% % % % % function [P_sup, P_wh4, x_dot] = BlocoHidraulicoLAC_FisicaRigorosa(PWM_LAC, CMD_MCV, CMD_PFV, CMD_IRL, CMD_ORL)
% % % % %     % #####################################################################
% % % % %     % MODELO HIDRÁULICO EAB REFINADO - COMPORTAMENTO NÃO-LINEAR (PSI)
% % % % %     % #####################################################################
% % % % % 
% % % % %     % --- PARÂMETROS CONSTANTES ---
% % % % %     dt = 0.001;                 % Passo de tempo (1 ms)
% % % % %     P_atm = 101325;             % Pressão atm (Pa)
% % % % %     P_max_pa = 190 * 1e5;       % Limite físico do sistema: 190 bar em Pascal
% % % % % 
% % % % %     % Parâmetros Geométricos do LAC
% % % % %     A_p = 2.85e-4;              % Área efetiva do pistão do LAC (m²)
% % % % %     K_drv = 2.69e-4;            % m/s por %PWM
% % % % %     x_max = 0.0537;             % Curso máximo do LAC (53.7 mm)
% % % % % 
% % % % %     % Parâmetros do Caliper 4 e Linha
% % % % %     D_caliper = 0.040;          % Diâmetro do pistão da pinça (40 mm)
% % % % %     A_caliper = pi*(D_caliper/2)^2; 
% % % % %     deadstroke_max = 0.005;     % Folga pastilha-disco (5 mm)
% % % % %     V_dead_max = A_caliper * deadstroke_max; % Volume do deadstroke (~6.28 mL)
% % % % %     V_line_dead = 5e-6;         % Volume morto da linha rígida isolada (5 mL)
% % % % % 
% % % % %     % Parâmetros de Restrição da Válvula Solenoide (65 cm³/s @ 25 bar)
% % % % %     Q_nom = 65e-6;              
% % % % %     dP_nom = 25e5;              
% % % % %     C_v = Q_nom / sqrt(dP_nom); 
% % % % % 
% % % % %     % --- VARIÁVEIS DE ESTADO (PERSISTENT) ---
% % % % %     persistent x_lac P_sup_state P_wh4_state V_to_caliper
% % % % %     if isempty(x_lac)
% % % % %         x_lac = 0.0;            % Posição inicial do LAC (m)
% % % % %         P_sup_state = P_atm;     % Pressão inicial de suprimento (Pa)
% % % % %         P_wh4_state = P_atm;     % Pressão inicial na roda (Pa)
% % % % %         V_to_caliper = 0.0;     % Volume acumulado enviado para a pinça (m³)
% % % % %     end
% % % % % 
% % % % %     % --- 1. DINÂMICA DE DESLOCAMENTO DO LAC (FIM DE CURSO RIGOROSO) ---
% % % % %     x_dot = 0.0;
% % % % %     if x_lac < x_max
% % % % %         x_dot = PWM_LAC * K_drv;
% % % % %         x_lac = x_lac + x_dot * dt;
% % % % %         if x_lac > x_max
% % % % %             x_lac = x_max;
% % % % %             x_dot = 0.0; % Parou no batente mecânico
% % % % %         end
% % % % %     end
% % % % %     Q_lac = A_p * x_dot; % Vazão volumétrica gerada pelo movimento
% % % % % 
% % % % %     % --- 2. LÓGICA DIGITAL DAS VÁLVULAS ---
% % % % %     open_MCV = (CMD_MCV == 0);
% % % % %     open_PFV = (CMD_PFV == 1);
% % % % %     open_IRL = (CMD_IRL == 0);
% % % % %     open_ORL = (CMD_ORL == 1);
% % % % % 
% % % % %     % --- 3. EQUAÇÕES DE ESCOAMENTO (BERNOULLI COM ACOPLAMENTO) ---
% % % % %     Q_irl = 0;
% % % % %     if open_IRL
% % % % %         dP_irl = P_sup_state - P_wh4_state;
% % % % %         Q_irl = C_v * sign(dP_irl) * sqrt(abs(dP_irl));
% % % % %     end
% % % % % 
% % % % %     Q_orl = 0;
% % % % %     if open_ORL
% % % % %         dP_orl = P_wh4_state - P_atm;
% % % % %         Q_orl = C_v * sign(dP_orl) * sqrt(abs(dP_orl));
% % % % %     end
% % % % % 
% % % % %     % --- 4. COMPRESSIBILIDADE E COMPLACÊNCIA NÃO-LINEAR (EFEITO EXPONENCIAL) ---
% % % % %     % Módulo de elasticidade dinâmico do fluido (varia com a pressão para simular rigidez)
% % % % %     Beta_fluid = 1.4e9; 
% % % % % 
% % % % %     % Dinâmica da Pressão de Suprimento (P_sup)
% % % % %     % NOTA: Se a IRL fechar, V_line_dead é minúsculo, fazendo a pressão disparar rápido!
% % % % %     dP_sup_dt = (Beta_fluid / V_line_dead) * (Q_lac - Q_irl);
% % % % %     P_sup_state = P_sup_state + dP_sup_dt * dt;
% % % % % 
% % % % %     % Dinâmica da Pressão de Roda (P_wh4) com Deadstroke e Rigidez de Pastilha
% % % % %     Q_net_wheel = Q_irl - Q_orl;
% % % % %     V_to_caliper = max(0, V_to_caliper + Q_net_wheel * dt);
% % % % % 
% % % % %     if V_to_caliper <= V_dead_max
% % % % %         % FASE 1: Consumindo os 5mm de Deadstroke. Pressão manométrica é ZERO.
% % % % %         P_wh4_state = P_atm;
% % % % %     else
% % % % %         % FASE 2: Contato com o disco. O volume excedente esmaga a mola não-linear da pastilha.
% % % % %         V_compressed = V_to_caliper - V_dead_max;
% % % % % 
% % % % %         % Função exponencial de rigidez: a pressão ganha curvatura com o esmagamento volumétrico
% % % % %         % Adota uma aproximação clássica de complacência de freios (p = k * V^1.5 ou exponencial)
% % % % %         P_gauge = 0.5e5 * (V_compressed / 1e-7)^1.8; 
% % % % %         P_wh4_state = P_atm + P_gauge;
% % % % %     end
% % % % % 
% % % % %     % --- 5. SATURAÇÃO FÍSICA E LIMITE DE 190 BAR ---
% % % % %     if P_sup_state > P_max_pa, P_sup_state = P_max_pa; end
% % % % %     if P_wh4_state > P_max_pa, P_wh4_state = P_max_pa; end
% % % % %     if P_sup_state < P_atm, P_sup_state = P_atm; end
% % % % %     if P_wh4_state < P_atm, P_wh4_state = P_atm; end
% % % % % 
% % % % %     % --- 6. CONVERSÃO FINAL DAS SAÍDAS PARA PSI ---
% % % % %     % 1 Pascal = 0.0001450377377 PSI
% % % % %     pa_to_psi = 1.450377e-4;
% % % % %     P_sup = (P_sup_state - P_atm) * pa_to_psi;
% % % % %     P_wh4 = (P_wh4_state - P_atm) * pa_to_psi;
% % % % % end
% % % % % % function [P_sup, P_wh4, x_dot] = hydraulic_block_EAB(PWM_LAC, CMD_MCV, CMD_PFV, CMD_IRL, CMD_ORL)
% % % % % %     % #####################################################################
% % % % % %     % MODELO DO BLOCO HIDRÁULICO EAB - CALIPER 4 (CAMINHO VERDE E AZUL)
% % % % % %     % Inputs:
% % % % % %     %   PWM_LAC : Sinal de comando do atuador linear (0 a 100%)
% % % % % %     %   CMD_MCV : Comando da Válvula de Controle do Cilindro Mestre (0=NO, 1=Fechada)
% % % % % %     %   CMD_PFV : Comando da Válvula de Alimentação do LAC (0=NC, 1=Aberta)
% % % % % %     %   CMD_IRL : Comando da Válvula de Entrada da Roda (0=NO, 1=Fechada)
% % % % % %     %   CMD_ORL : Comando da Válvula de Saída da Roda (0=NC, 1=Aberta)
% % % % % %     % #####################################################################
% % % % % % 
% % % % % %     % --- PARÂMETROS CONSTANTES DO SISTEMA ---
% % % % % %     dt = 0.001;                 % Passo de tempo da simulação (1 ms)
% % % % % %     Beta = 1.4e9;               % Bulk Modulus do fluido de freio (Pa)
% % % % % %     P_atm = 101325;             % Pressão atmosférica/reservatório (Pa)
% % % % % %     rho = 900;                  % Densidade do fluido de freio (kg/m³)
% % % % % % 
% % % % % %     % Parâmetros do LAC
% % % % % %     A_p = 2.85e-4;              % Área efetiva do pistão do LAC (m²)
% % % % % %     K_drv = 2.69e-4;            % Ganho de velocidade do pistão (m/s por %PWM)
% % % % % % 
% % % % % %     % Parâmetros do Caliper 4
% % % % % %     D_caliper = 0.040;          % ASSUMIDO: Diâmetro do pistão da pinça (40 mm = 0.04 m)
% % % % % %     A_caliper = pi*(D_caliper/2)^2; % Área do pistão da pinça (m²)
% % % % % %     deadstroke_max = 0.005;     % Folga pastilha-disco (5 mm = 0.005 m)
% % % % % %     V_dead_max = A_caliper * deadstroke_max; % Volume morto máximo (m³)
% % % % % %     V_line = 10e-6;             % ASSUMIDO: Volume da linha hidráulica (10 mL)
% % % % % % 
% % % % % %     % Parâmetros das Válvulas (Nominal: 65 cm³/s @ 25 bar)
% % % % % %     Q_nom = 65e-6;              % Vazão nominal (m³/s)
% % % % % %     dP_nom = 25e5;              % Diferença de pressão nominal (Pa)
% % % % % %     C_v = Q_nom / sqrt(dP_nom); % Coeficiente de restrição calculado
% % % % % % 
% % % % % %     % --- VARIÁVEIS DE ESTADO (PERSISTENT) ---
% % % % % %     persistent P_sup_state P_wh4_state V_dead_consumed
% % % % % %     if isempty(P_sup_state)
% % % % % %         P_sup_state = P_atm;     % Pressão inicial de suprimento (Pascal)
% % % % % %         P_wh4_state = P_atm;     % Pressão inicial na roda (Pascal)
% % % % % %         V_dead_consumed = 0.0;   % Volume consumido no deslocamento da pastilha
% % % % % %     end
% % % % % % 
% % % % % %     % --- 1. DINÂMICA DO ATUADOR LAC ---
% % % % % %     % Velocidade e vazão volumétrica gerada pelo LAC
% % % % % %     x_dot = PWM_LAC * K_drv;
% % % % % %     Q_lac = A_p * x_dot;
% % % % % % 
% % % % % %     % --- 2. LÓGICA DIGITAL DAS VÁLVULAS (NO / NC) ---
% % % % % %     % MCV (Normalmente Aberta)
% % % % % %     if CMD_MCV == 0, open_MCV = 1; else, open_MCV = 0; end
% % % % % %     % PFV (Normalmente Fechada)
% % % % % %     if CMD_PFV == 1, open_PFV = 1; else, open_PFV = 0; end
% % % % % %     % IRL (Normalmente Aberta)
% % % % % %     if CMD_IRL == 0, open_IRL = 1; else, open_IRL = 0; end
% % % % % %     % ORL (Normalmente Fechada)
% % % % % %     if CMD_ORL == 1, open_ORL = 1; else, open_ORL = 0; end
% % % % % % 
% % % % % %     % --- 3. CÁLCULO DAS VAZÕES ENTRE CÂMARAS ---
% % % % % %     % Vazão pela PFV (Suprimento LAC -> Nó Central do Caminho Verde)
% % % % % %     % Se fechada, a vazão é zero. Se aberta, depende do gradiente de pressão.
% % % % % %     Q_pfv = 0;
% % % % % %     if open_PFV == 1
% % % % % %         dP_pfv = P_sup_state - P_atm; % Alimentação vinda do reservatório/acumulador
% % % % % %         Q_pfv = C_v * sign(dP_pfv) * sqrt(abs(dP_pfv));
% % % % % %     end
% % % % % % 
% % % % % %     % Vazão de Entrada na Roda 4 via IRL (Caminho Verde -> Caliper 4)
% % % % % %     Q_irl = 0;
% % % % % %     if open_IRL == 1
% % % % % %         dP_irl = P_sup_state - P_wh4_state;
% % % % % %         Q_irl = C_v * sign(dP_irl) * sqrt(abs(dP_irl));
% % % % % %     end
% % % % % % 
% % % % % %     % Vazão de Saída da Roda 4 via ORL (Caliper 4 -> Linha de Retorno Azul)
% % % % % %     Q_orl = 0;
% % % % % %     if open_ORL == 1
% % % % % %         dP_orl = P_wh4_state - P_atm; % Retorno direto para o reservatório (Caminho Azul)
% % % % % %         Q_orl = C_v * sign(dP_orl) * sqrt(abs(dP_orl));
% % % % % %     end
% % % % % % 
% % % % % %     % --- 4. BALANÇO DE PRESSÃO E CONSUMO DE DEADSTROKE ---
% % % % % % 
% % % % % %     % Atualização da Pressão de Suprimento (Nó do LAC)
% % % % % %     % O acúmulo de pressão depende do escoamento gerado e do que sai pelas válvulas
% % % % % %     dP_sup_dt = (Beta / V_line) * (Q_lac - Q_irl);
% % % % % %     P_sup_state = P_sup_state + dP_sup_dt * dt;
% % % % % %     if P_sup_state < P_atm, P_sup_state = P_atm; end % Saturação física
% % % % % % 
% % % % % %     % Dinâmica da Roda 4 (Caliper) incorporando o Deadstroke
% % % % % %     Q_net_wheel = Q_irl - Q_orl;
% % % % % % 
% % % % % %     if V_dead_consumed < V_dead_max && Q_net_wheel > 0
% % % % % %         % Fase de aproximação: Consome o volume morto, pressão não sobe significativamente
% % % % % %         V_dead_consumed = V_dead_consumed + Q_net_wheel * dt;
% % % % % %         dP_wh4_dt = 0; 
% % % % % %         P_wh4_state = P_atm; % Mantém em pressão manométrica zero
% % % % % %     elseif V_dead_consumed >= V_dead_max
% % % % % %         % Fase de contato: Pastilha encostou no disco, pressão sobe rigidamente
% % % % % %         dP_wh4_dt = (Beta / V_line) * Q_net_wheel;
% % % % % %         P_wh4_state = P_wh4_state + dP_wh4_dt * dt;
% % % % % %     else
% % % % % %         % Caso haja alívio de pressão e retorno da pastilha
% % % % % %         if P_wh4_state > P_atm
% % % % % %             dP_wh4_dt = (Beta / V_line) * Q_net_wheel;
% % % % % %             P_wh4_state = P_wh4_state + dP_wh4_dt * dt;
% % % % % %         else
% % % % % %             P_wh4_state = P_atm;
% % % % % %             V_dead_consumed = max(0, V_dead_consumed + Q_net_wheel * dt);
% % % % % %             dP_wh4_dt = 0;
% % % % % %         end
% % % % % %     end
% % % % % % 
% % % % % %     % Saturação inferior de segurança física
% % % % % %     if P_wh4_state < P_atm, P_wh4_state = P_atm; end
% % % % % % 
% % % % % %     % --- 5. CONVERSÃO PARA UNIDADE COMUM (PSI) ---
% % % % % %     P_sup = (P_sup_state - P_atm) / 1.45038e-4;
% % % % % %     P_wh4 = (P_wh4_state - P_atm) / 1.45038e-4;
% % % % % % end
% % % % % % 
% % % % % % % function [Psup_dot, Pw_dot, x_dot, Qlac, Qmcv, Qin, Qout] = BlocoHidraulicoLAC( ...
% % % % % % %     u_pwm, mcv_open, pfv_open, irl_open, orl_open, Psup, Pw, x)
% % % % % % % % Modelo hidráulico MK C2 (EAB/ACC) — nó de suprimento (Psup) e roda/caliper (Pw)
% % % % % % % % Convenção: 1 = válvula ABERTA (mcv_open, pfv_open, irl_open, orl_open)
% % % % % % % % Saídas: derivadas Psup_dot, Pw_dot, x_dot e vazões Qlac, Qmcv, Qin, Qout
% % % % % % % % Unidades internas: SI (Pa, m, m^3/s, kg/m^3). Pressões são ABSOLUTAS.
% % % % % % % 
% % % % % % % % ===== Fluido / referências =====
% % % % % % % rho    = 850;           % kg/m^3 (DOT típico)
% % % % % % % P_atm  = 1.01325e5;     % Pa
% % % % % % % Pret   = P_atm;         % reservatório (referência)
% % % % % % % DP_MIN = 500;           % Pa — faixa morta para ΔP ~ 0 (evita ruído numérico)
% % % % % % % 
% % % % % % % % ===== Geometria LAC (MK C2) =====
% % % % % % % D_mc   = 19.05e-3;                  % m (êmbolo master)
% % % % % % % A_p    = pi*(D_mc/2)^2;             % m^2 (~2.85e-4)
% % % % % % % V_t    = 15.3e-6;                   % m^3 (15.3 mL) volume deslocável
% % % % % % % x_max  = V_t / A_p;                 % m (~0.0537 m)
% % % % % % % 
% % % % % % % % ===== Driver do fuso (MK C2) =====
% % % % % % % mm_per_rev = 42.63/73;              % mm/rev
% % % % % % % m_per_rev  = mm_per_rev * 1e-3;     % m/rev
% % % % % % % f_max_hz   = 46;                    % rev/s
% % % % % % % K_drv      = (f_max_hz * m_per_rev) / 100;  % (m/s)/%PWM
% % % % % % % 
% % % % % % % % ===== Volumes efetivos (ajustáveis por aplicação) =====
% % % % % % % V0_sup = 6.0e-5;      % m^3 (manifold/suprimento ~ 60 mL)
% % % % % % % Vw     = 1.0e-5;      % m^3 (linha+caliper roda ~ 10 mL)
% % % % % % % V_min  = 1.0e-6;      % m^3 (proteção numérica)
% % % % % % % 
% % % % % % % % ===== Chaves de modelo =====
% % % % % % % USE_BETA_VAR = true;    % true: β(P) variável (ar+fluido); false: β constante
% % % % % % % USE_VVAR     = true;    % true: Vsup(x) = V0_sup − A_p*x; false: Vsup constante
% % % % % % % 
% % % % % % % % ===== β constante (validação) =====
% % % % % % % beta_const = 0.08e9;    % Pa (≈80 MPa efetivo)
% % % % % % % 
% % % % % % % % ===== β(P) variável (realismo com ar) =====
% % % % % % % beta_liq = 1.5e9;       % Pa (fluido puro)
% % % % % % % eps0     = 0.03;        % fração volumétrica de ar a 1 atm (2–6% típico)
% % % % % % % gamma_ar = 1.4;         % razão de calores específicos do ar
% % % % % % % 
% % % % % % % % ===== Válvulas (lei do orifício) =====
% % % % % % % Cv   = 0.62;            % coeficiente de descarga
% % % % % % % Amcv = 3.0e-6;          % m^2 (MCV)
% % % % % % % Airl = 3.0e-7;          % m^2 (IRL)
% % % % % % % Aorl = 3.0e-7;          % m^2 (ORL)
% % % % % % % 
% % % % % % % % ===== Vazamentos opcionais (fechamento de balanço) =====
% % % % % % % K_leak_sup = 0.0;       % m^3/(s·Pa) — vazamento Psup→reservatório (default 0)
% % % % % % % K_leak_w   = 0.0;       % m^3/(s·Pa) — vazamento Pw→reservatório (default 0)
% % % % % % % 
% % % % % % % % ===== Sanitização das entradas =====
% % % % % % % u_pwm    = max(min(u_pwm, 100), -100);
% % % % % % % mcv_open = double(mcv_open ~= 0);
% % % % % % % pfv_open = double(pfv_open ~= 0);
% % % % % % % irl_open = double(irl_open ~= 0);
% % % % % % % orl_open = double(orl_open ~= 0);
% % % % % % % Psup     = max(Psup, Pret);   % absolutas ≥ pressão do reservatório
% % % % % % % Pw       = max(Pw,   Pret);
% % % % % % % x        = min(max(x, 0), x_max);
% % % % % % % 
% % % % % % % % ===== Cinemática do êmbolo (saturada no curso) =====
% % % % % % % v_cmd = K_drv * u_pwm;               % m/s
% % % % % % % if (x <= 0 && v_cmd < 0)
% % % % % % %     x_dot = 0;
% % % % % % % elseif (x >= x_max && v_cmd > 0)
% % % % % % %     x_dot = 0;
% % % % % % % else
% % % % % % %     x_dot = v_cmd;
% % % % % % % end
% % % % % % % 
% % % % % % % % ===== Vazão do LAC (PFV como chave) =====
% % % % % % % Qlac = pfv_open * A_p * x_dot;       % m^3/s
% % % % % % % 
% % % % % % % % ===== Orifícios com proteção numérica (faixa morta ΔP) =====
% % % % % % % % MCV: Psup ↔ Pret
% % % % % % % dP_mcv = Psup - Pret;
% % % % % % % if abs(dP_mcv) < DP_MIN
% % % % % % %     Qmcv = 0;
% % % % % % % else
% % % % % % %     Qmcv = mcv_open * Cv * Amcv * sign(dP_mcv) * sqrt(2 * abs(dP_mcv) / rho);
% % % % % % % end
% % % % % % % 
% % % % % % % % IRL: Psup ↔ Pw
% % % % % % % dP_irl = Psup - Pw;
% % % % % % % if abs(dP_irl) < DP_MIN
% % % % % % %     Qin = 0;
% % % % % % % else
% % % % % % %     Qin = irl_open * Cv * Airl * sign(dP_irl) * sqrt(2 * abs(dP_irl) / rho);
% % % % % % % end
% % % % % % % 
% % % % % % % % ORL: Pw ↔ Pret
% % % % % % % dP_orl = Pw - Pret;
% % % % % % % if abs(dP_orl) < DP_MIN
% % % % % % %     Qout = 0;
% % % % % % % else
% % % % % % %     Qout = orl_open * Cv * Aorl * sign(dP_orl) * sqrt(2 * abs(dP_orl) / rho);
% % % % % % % end
% % % % % % % 
% % % % % % % % Vazamentos (lineares em ΔP para simplicidade)
% % % % % % % Qleak_sup = K_leak_sup * max(Psup - Pret, 0);   % Psup → reservatório
% % % % % % % Qleak_w   = K_leak_w   * max(Pw   - Pret, 0);   % Pw   → reservatório
% % % % % % % 
% % % % % % % % ===== Volumes (variável no suprimento) =====
% % % % % % % if USE_VVAR
% % % % % % %     Vsup = max(V0_sup - A_p * x, V_min);
% % % % % % % else
% % % % % % %     Vsup = V0_sup;
% % % % % % % end
% % % % % % % 
% % % % % % % % ===== Compressibilidade efetiva =====
% % % % % % % if USE_BETA_VAR
% % % % % % %     % Pressões absolutas para o modelo de ar
% % % % % % %     P_sup_abs = max(Psup, P_atm + 1);
% % % % % % %     P_w_abs   = max(Pw,   P_atm + 1);
% % % % % % % 
% % % % % % %     % fração de ar à pressão atual
% % % % % % %     eps_sup = eps0 * (P_atm / P_sup_abs)^(1 / gamma_ar);
% % % % % % %     eps_w   = eps0 * (P_atm / P_w_abs  )^(1 / gamma_ar);
% % % % % % % 
% % % % % % %     % bulk modulus efetivo
% % % % % % %     beta_sup = 1.0 / (1.0 / beta_liq + eps_sup / (gamma_ar * P_sup_abs));
% % % % % % %     beta_w   = 1.0 / (1.0 / beta_liq + eps_w   / (gamma_ar * P_w_abs));
% % % % % % % else
% % % % % % %     beta_sup = beta_const;
% % % % % % %     beta_w   = beta_const;
% % % % % % % end
% % % % % % % 
% % % % % % % % ===== Dinâmica das pressões =====
% % % % % % % % Balanços de vazão:
% % % % % % % %  Suprimento: entra Qlac; sai Qmcv, Qin, vazamento Qleak_sup
% % % % % % % %  Roda:       entra Qin;  sai Qout, vazamento Qleak_w
% % % % % % % Psup_dot = (beta_sup / Vsup) * (Qlac - Qmcv - Qin - Qleak_sup);
% % % % % % % Pw_dot   = (beta_w   / Vw  ) * (Qin  - Qout - Qleak_w);
% % % % % % % 
% % % % % % % end
% % % % % % % % function [Psup_dot, Pw_dot, x_dot, Qlac, Qmcv, Qin, Qout] = BlocoHidraulicoLAC(u_pwm, mcv_open, pfv_open, irl_open, orl_open, Psup, Pw, x)
% % % % % % % % % Modelo hidráulico LAC – 1=valvula aberta (mcv_open, pfv_open, irl_open, orl_open)
% % % % % % % % % Saídas: derivadas Psup_dot, Pw_dot, x_dot e vazões Qlac, Qmcv, Qin, Qout
% % % % % % % % 
% % % % % % % % % ----- Parâmetros do fluido -----
% % % % % % % % rho   = 850;           % kg/m^3
% % % % % % % % P_atm = 1.01325e5;     % Pa
% % % % % % % % Pret  = P_atm;
% % % % % % % % 
% % % % % % % % % ----- Geometria do LAC -----
% % % % % % % % D_mc  = 19.05e-3;                    % m
% % % % % % % % A_p   = pi*(D_mc/2)^2;               % m^2
% % % % % % % % V_t   = 15.3e-6;                     % m^3
% % % % % % % % x_max = V_t / A_p;                   % m
% % % % % % % % 
% % % % % % % % % ----- Driver do fuso -----
% % % % % % % % mm_per_rev = 42.63/73;               % mm/rev
% % % % % % % % m_per_rev  = mm_per_rev * 1e-3;      % m/rev
% % % % % % % % f_max_hz   = 46;                     % Hz
% % % % % % % % K_drv      = f_max_hz * m_per_rev / 100;  % (m/s)/%PWM
% % % % % % % % 
% % % % % % % % % ----- Volumes -----
% % % % % % % % V0_sup = 6.0e-5;      % m^3 (manifold/suprimento)
% % % % % % % % Vw     = 1.0e-5;      % m^3 (roda/caliper)
% % % % % % % % V_min  = 1.0e-6;      % m^3 (limite numérico)
% % % % % % % % 
% % % % % % % % % ----- Chaves de modelo -----
% % % % % % % % USE_BETA_VAR = true;  % true = beta(P) variável; false = beta constante
% % % % % % % % USE_VVAR     = true;  % true = Vsup(x) variável; false = Vsup constante
% % % % % % % % 
% % % % % % % % % ----- beta constante (validação) -----
% % % % % % % % beta_const = 0.08e9;  % Pa
% % % % % % % % 
% % % % % % % % % ----- beta(P) variável (realismo) -----
% % % % % % % % beta_liq = 1.5e9;     % Pa
% % % % % % % % eps0     = 0.03;      % fração de ar a 1 atm (ajuste)
% % % % % % % % gamma_ar = 1.4;
% % % % % % % % 
% % % % % % % % % ----- Válvulas -----
% % % % % % % % Cv   = 0.62;
% % % % % % % % Amcv = 3.0e-6;        % m^2
% % % % % % % % Airl = 3.0e-7;        % m^2
% % % % % % % % Aorl = 3.0e-7;        % m^2
% % % % % % % % 
% % % % % % % % % ----- Sanitização -----
% % % % % % % % u_pwm    = max(min(u_pwm,100),-100);
% % % % % % % % mcv_open = double(mcv_open ~= 0);
% % % % % % % % pfv_open = double(pfv_open ~= 0);
% % % % % % % % irl_open = double(irl_open ~= 0);
% % % % % % % % orl_open = double(orl_open ~= 0);
% % % % % % % % Psup     = max(Psup, Pret);
% % % % % % % % Pw       = max(Pw,   Pret);
% % % % % % % % x        = min(max(x, 0), x_max);
% % % % % % % % 
% % % % % % % % % ----- Cinemática do pistão -----
% % % % % % % % v_cmd = K_drv * u_pwm;
% % % % % % % % if (x <= 0 && v_cmd < 0)
% % % % % % % %     x_dot = 0;
% % % % % % % % elseif (x >= x_max && v_cmd > 0)
% % % % % % % %     x_dot = 0;
% % % % % % % % else
% % % % % % % %     x_dot = v_cmd;
% % % % % % % % end
% % % % % % % % 
% % % % % % % % % ----- Vazões -----
% % % % % % % % Qlac = pfv_open * A_p * x_dot;
% % % % % % % % 
% % % % % % % % dP_mcv = Psup - Pret;
% % % % % % % % Qmcv   = mcv_open * Cv * Amcv * sign(dP_mcv) * sqrt(2 * abs(dP_mcv) / rho);
% % % % % % % % 
% % % % % % % % dP_irl = Psup - Pw;
% % % % % % % % Qin    = irl_open * Cv * Airl * sign(dP_irl) * sqrt(2 * abs(dP_irl) / rho);
% % % % % % % % 
% % % % % % % % dP_orl = Pw - Pret;
% % % % % % % % Qout   = orl_open * Cv * Aorl * sign(dP_orl) * sqrt(2 * abs(dP_orl) / rho);
% % % % % % % % 
% % % % % % % % % ----- Volumes -----
% % % % % % % % if USE_VVAR
% % % % % % % %     Vsup = max(V0_sup - A_p * x, V_min);
% % % % % % % % else
% % % % % % % %     Vsup = V0_sup;
% % % % % % % % end
% % % % % % % % 
% % % % % % % % % ----- beta efetivo -----
% % % % % % % % if USE_BETA_VAR
% % % % % % % %     P_sup_abs = max(Psup, P_atm + 1);
% % % % % % % %     P_w_abs   = max(Pw,   P_atm + 1);
% % % % % % % %     eps_sup   = eps0 * (P_atm / P_sup_abs)^(1 / gamma_ar);
% % % % % % % %     eps_w     = eps0 * (P_atm / P_w_abs  )^(1 / gamma_ar);
% % % % % % % %     beta_sup  = 1 / (1 / beta_liq + eps_sup / (gamma_ar * P_sup_abs));
% % % % % % % %     beta_w    = 1 / (1 / beta_liq + eps_w   / (gamma_ar * P_w_abs));
% % % % % % % % else
% % % % % % % %     beta_sup  = beta_const;
% % % % % % % %     beta_w    = beta_const;
% % % % % % % % end
% % % % % % % % 
% % % % % % % % % ----- Dinâmica das pressões -----
% % % % % % % % Psup_dot = (beta_sup / Vsup) * (Qlac - Qmcv - Qin);
% % % % % % % % Pw_dot   = (beta_w   / Vw  ) * (Qin  - Qout);
% % % % % % % % end
% % % % % % % % 
% % % % % % % % % function [Psup_dot, Pw_dot, x_dot, Qlac, Qmcv, Qin, Qout] = BlocoHidraulicoLAC( ...
% % % % % % % % %     u_pwm, mcv, pfv, irl, orl, Psup, Pw, x)
% % % % % % % % % % ---------------------------------------------------------------
% % % % % % % % % % Modelo hidráulico LAC — β(P) variável + volume variável
% % % % % % % % % % ---------------------------------------------------------------
% % % % % % % % % 
% % % % % % % % % % ========== FLUIDO ==========
% % % % % % % % % beta_liq = 1.5e9;      % Pa — bulk modulus do fluido puro (sem ar)
% % % % % % % % % eps0     = 0.03;        % fração de ar a P_atm (3% — ajustar ao sistema)
% % % % % % % % % gamma_ar = 1.4;         % razão de calores específicos do ar
% % % % % % % % % P_atm    = 1.01325e5;   % Pa
% % % % % % % % % rho      = 850;         % kg/m³
% % % % % % % % % Pret     = P_atm;       % pressão do reservatório
% % % % % % % % % 
% % % % % % % % % % ========== GEOMETRIA DO LAC ==========
% % % % % % % % % D_mc  = 19.05e-3;
% % % % % % % % % A_p   = pi * (D_mc/2)^2;
% % % % % % % % % V_t   = 15.3e-6;
% % % % % % % % % x_max = V_t / A_p;
% % % % % % % % % 
% % % % % % % % % % ========== DRIVER DO FUSO ==========
% % % % % % % % % mm_per_rev = 42.63 / 73;
% % % % % % % % % m_per_rev  = mm_per_rev * 1e-3;
% % % % % % % % % f_max_hz   = 46;
% % % % % % % % % K_drv      = f_max_hz * m_per_rev / 100;
% % % % % % % % % 
% % % % % % % % % % ========== VOLUMES DE CONTROLE ==========
% % % % % % % % % V0_sup = 6.0e-5;
% % % % % % % % % V0_w   = 1.0e-5;
% % % % % % % % % V_min  = 1.0e-6;
% % % % % % % % % 
% % % % % % % % % Vsup = max(V0_sup - A_p * x, V_min);
% % % % % % % % % Vw   = V0_w;
% % % % % % % % % 
% % % % % % % % % % ========== β EFETIVO = f(P) ==========
% % % % % % % % % %
% % % % % % % % % %  À medida que P sobe, o ar comprime, β cresce, dP/dt acelera
% % % % % % % % % %  ISSO gera a curva exponencial
% % % % % % % % % %
% % % % % % % % % P_sup_abs = max(Psup, P_atm + 1);   % evita divisão por ~0
% % % % % % % % % P_w_abs   = max(Pw,   P_atm + 1);
% % % % % % % % % 
% % % % % % % % % % Fração de ar à pressão atual
% % % % % % % % % eps_sup = eps0 * (P_atm / P_sup_abs)^(1/gamma_ar);
% % % % % % % % % eps_w   = eps0 * (P_atm / P_w_abs  )^(1/gamma_ar);
% % % % % % % % % 
% % % % % % % % % % Bulk modulus efetivo
% % % % % % % % % beta_sup = 1.0 / (1.0/beta_liq + eps_sup/(gamma_ar * P_sup_abs));
% % % % % % % % % beta_w   = 1.0 / (1.0/beta_liq + eps_w  /(gamma_ar * P_w_abs));
% % % % % % % % % 
% % % % % % % % % % ========== VÁLVULAS ==========
% % % % % % % % % Cv   = 0.62;
% % % % % % % % % Amcv = 3.0e-6;
% % % % % % % % % Airl = 3.0e-7;
% % % % % % % % % Aorl = 3.0e-7;
% % % % % % % % % 
% % % % % % % % % % ========== SANITIZAÇÃO ==========
% % % % % % % % % u_pwm = max(min(u_pwm, 100), -100);
% % % % % % % % % mcv   = double(mcv ~= 0);
% % % % % % % % % pfv   = double(pfv ~= 0);
% % % % % % % % % irl   = double(irl ~= 0);
% % % % % % % % % orl   = double(orl ~= 0);
% % % % % % % % % Psup  = max(Psup, Pret);
% % % % % % % % % Pw    = max(Pw,   Pret);
% % % % % % % % % x     = max(min(x, x_max), 0);
% % % % % % % % % 
% % % % % % % % % % ========== CINEMÁTICA ==========
% % % % % % % % % v_cmd = K_drv * u_pwm;
% % % % % % % % % 
% % % % % % % % % if (x <= 0 && v_cmd < 0)
% % % % % % % % %     x_dot = 0;
% % % % % % % % % elseif (x >= x_max && v_cmd > 0)
% % % % % % % % %     x_dot = 0;
% % % % % % % % % else
% % % % % % % % %     x_dot = v_cmd;
% % % % % % % % % end
% % % % % % % % % 
% % % % % % % % % % ========== VAZÕES ==========
% % % % % % % % % Qlac = pfv * A_p * x_dot;
% % % % % % % % % 
% % % % % % % % % dP_mcv = Psup - Pret;
% % % % % % % % % Qmcv   = mcv * Cv * Amcv * sign(dP_mcv) * sqrt(2 * abs(dP_mcv) / rho);
% % % % % % % % % 
% % % % % % % % % dP_irl = Psup - Pw;
% % % % % % % % % Qin    = irl * Cv * Airl * sign(dP_irl) * sqrt(2 * abs(dP_irl) / rho);
% % % % % % % % % 
% % % % % % % % % dP_orl = Pw - Pret;
% % % % % % % % % Qout   = orl * Cv * Aorl * sign(dP_orl) * sqrt(2 * abs(dP_orl) / rho);
% % % % % % % % % 
% % % % % % % % % % ========== EQUAÇÕES DE ESTADO ==========
% % % % % % % % % %
% % % % % % % % % %  Agora β = f(P): começa baixo → cresce com P → dP/dt acelera
% % % % % % % % % %
% % % % % % % % % Psup_dot = (beta_sup / Vsup) * (Qlac - Qmcv - Qin);
% % % % % % % % % Pw_dot   = (beta_w   / Vw)   * (Qin  - Qout);
% % % % % % % % % 
% % % % % % % % % end
% % % % % % % % % % function [Psup_dot, Pw_dot, x_dot, Qlac, Qmcv, Qin, Qout] = BlocoHidraulicoLAC( ...
% % % % % % % % % %     u_pwm, mcv, pfv, irl, orl, Psup, Pw, x)
% % % % % % % % % % % ---------------------------------------------------------------
% % % % % % % % % % % Modelo hidráulico LAC — volumes de controle com compressibilidade
% % % % % % % % % % % 3 estados: x, Psup, Pw
% % % % % % % % % % % ---------------------------------------------------------------
% % % % % % % % % % 
% % % % % % % % % % % ========== PARÂMETROS DO FLUIDO ==========
% % % % % % % % % % beta_eff = 0.08e9;     % Pa — módulo efetivo (inclui ar, mangueiras)
% % % % % % % % % % rho      = 850;        % kg/m³
% % % % % % % % % % Pret     = 1e5;        % Pa — pressão do reservatório
% % % % % % % % % % 
% % % % % % % % % % % ========== GEOMETRIA DO LAC ==========
% % % % % % % % % % D_mc  = 19.05e-3;                  % m
% % % % % % % % % % A_p   = pi * (D_mc/2)^2;           % m² (~2.85e-4)
% % % % % % % % % % V_t   = 15.3e-6;                   % m³ — volume total deslocável
% % % % % % % % % % x_max = V_t / A_p;                 % m  — curso máximo (~53.7 mm)
% % % % % % % % % % 
% % % % % % % % % % % ========== DRIVER DO FUSO ==========
% % % % % % % % % % mm_per_rev = 42.63 / 73;           % mm/rev
% % % % % % % % % % m_per_rev  = mm_per_rev * 1e-3;    % m/rev
% % % % % % % % % % f_max_hz   = 46;                   % Hz
% % % % % % % % % % K_drv      = f_max_hz * m_per_rev / 100;  % (m/s) / %PWM
% % % % % % % % % % 
% % % % % % % % % % % ========== VOLUMES DE CONTROLE ==========
% % % % % % % % % % V0_sup = 6.0e-5;       % m³ — volume inicial do manifold
% % % % % % % % % % V0_w   = 1.0e-5;       % m³ — volume da roda/caliper
% % % % % % % % % % V_min  = 1.0e-6;       % m³ — limite inferior (evita div/0)
% % % % % % % % % % 
% % % % % % % % % % % Volume variável: pistão avança → volume livre diminui
% % % % % % % % % % Vsup = max(V0_sup - A_p * x, V_min);
% % % % % % % % % % Vw   = V0_w;
% % % % % % % % % % 
% % % % % % % % % % % ========== VÁLVULAS (lei do orifício) ==========
% % % % % % % % % % Cv = 0.62;             % coeficiente de descarga
% % % % % % % % % % 
% % % % % % % % % % % Áreas efetivas quando abertas
% % % % % % % % % % Amcv = 3.0e-6;         % m² — MCV (grande, baixa impedância)
% % % % % % % % % % Airl = 3.0e-7;         % m² — IRL
% % % % % % % % % % Aorl = 3.0e-7;         % m² — ORL
% % % % % % % % % % 
% % % % % % % % % % % ========== SANITIZAÇÃO ==========
% % % % % % % % % % u_pwm = max(min(u_pwm, 100), -100);
% % % % % % % % % % mcv   = double(mcv ~= 0);
% % % % % % % % % % pfv   = double(pfv ~= 0);
% % % % % % % % % % irl   = double(irl ~= 0);
% % % % % % % % % % orl   = double(orl ~= 0);
% % % % % % % % % % Psup  = max(Psup, Pret);
% % % % % % % % % % Pw    = max(Pw,   Pret);
% % % % % % % % % % x     = max(min(x, x_max), 0);
% % % % % % % % % % 
% % % % % % % % % % % ========== CINEMÁTICA DO PISTÃO ==========
% % % % % % % % % % v_cmd = K_drv * u_pwm;
% % % % % % % % % % 
% % % % % % % % % % if (x <= 0 && v_cmd < 0)
% % % % % % % % % %     x_dot = 0;
% % % % % % % % % % elseif (x >= x_max && v_cmd > 0)
% % % % % % % % % %     x_dot = 0;
% % % % % % % % % % else
% % % % % % % % % %     x_dot = v_cmd;
% % % % % % % % % % end
% % % % % % % % % % 
% % % % % % % % % % % ========== VAZÕES ==========
% % % % % % % % % % 
% % % % % % % % % % % LAC → suprimento (PFV como chave, não como restrição)
% % % % % % % % % % Qlac = pfv * A_p * x_dot;
% % % % % % % % % % 
% % % % % % % % % % % MCV: suprimento → reservatório
% % % % % % % % % % dP_mcv = Psup - Pret;
% % % % % % % % % % Qmcv   = mcv * Cv * Amcv * sign(dP_mcv) * sqrt(2 * abs(dP_mcv) / rho);
% % % % % % % % % % 
% % % % % % % % % % % IRL: suprimento → roda
% % % % % % % % % % dP_irl = Psup - Pw;
% % % % % % % % % % Qin    = irl * Cv * Airl * sign(dP_irl) * sqrt(2 * abs(dP_irl) / rho);
% % % % % % % % % % 
% % % % % % % % % % % ORL: roda → reservatório
% % % % % % % % % % dP_orl = Pw - Pret;
% % % % % % % % % % Qout   = orl * Cv * Aorl * sign(dP_orl) * sqrt(2 * abs(dP_orl) / rho);
% % % % % % % % % % 
% % % % % % % % % % % ========== EQUAÇÕES DE ESTADO ==========
% % % % % % % % % % %
% % % % % % % % % % %  dP/dt = (β_eff / V(x)) × ΣQ
% % % % % % % % % % %
% % % % % % % % % % %  Vsup diminui com x → dP/dt cresce → curva exponencial
% % % % % % % % % % %
% % % % % % % % % % Psup_dot = (beta_eff / Vsup) * (Qlac - Qmcv - Qin);
% % % % % % % % % % Pw_dot   = (beta_eff / Vw)   * (Qin  - Qout);
% % % % % % % % % % 
% % % % % % % % % % end
% % % % % % % % % % % function [Psup_dot, Pw_dot, x_dot, Qlac, Qmcv, Qin, Qout] = Bloco_Hidraulico_LAC( ...
% % % % % % % % % % %     u_pwm, mcv, pfv, irl, orl, Psup, Pw, x)
% % % % % % % % % % % 
% % % % % % % % % % % % ---------- fluido / retorno ----------
% % % % % % % % % % % beta = 0.08e9;         % Pa (efetivo, ajustado ao sistema real)
% % % % % % % % % % % rho  = 850;            % kg/m^3
% % % % % % % % % % % Pret = 1e5;            % Pa
% % % % % % % % % % % 
% % % % % % % % % % % % ---------- LAC ----------
% % % % % % % % % % % D_mc  = 19.05e-3;
% % % % % % % % % % % A_p   = pi*(D_mc/2)^2;
% % % % % % % % % % % V_t   = 15.3e-6;
% % % % % % % % % % % x_max = V_t / A_p;
% % % % % % % % % % % 
% % % % % % % % % % % % ---------- VOLUMES VARIÁVEIS (correção principal) ----------
% % % % % % % % % % % % Volume inicial total do circuito (suprimento + roda)
% % % % % % % % % % % V0_sup = 6.0e-5;       % m^3 - volume inicial do manifold/suprimento
% % % % % % % % % % % V0_w   = 1.0e-5;       % m^3 - volume inicial da roda/caliper
% % % % % % % % % % % V_min  = 1.0e-6;       % m^3 - volume mínimo (evita divisão por zero)
% % % % % % % % % % % 
% % % % % % % % % % % % O pistão do LAC reduz o volume livre do suprimento ao avançar
% % % % % % % % % % % Vsup = max(V0_sup - A_p * x, V_min);
% % % % % % % % % % % Vw   = V0_w;           % volume da roda é fixo (caliper rígido)
% % % % % % % % % % % 
% % % % % % % % % % % % ---------- Driver fuso ----------
% % % % % % % % % % % mm_per_rev = 42.63/73;
% % % % % % % % % % % m_per_rev  = mm_per_rev * 1e-3;
% % % % % % % % % % % f_max_hz   = 46;
% % % % % % % % % % % v_max_m_s  = f_max_hz * m_per_rev;
% % % % % % % % % % % K_drv      = v_max_m_s / 100;
% % % % % % % % % % % 
% % % % % % % % % % % % ---------- Válvulas ----------
% % % % % % % % % % % Cv = 0.62;
% % % % % % % % % % % Amcv_max = 3.0e-6;
% % % % % % % % % % % Apfv_max = 3.0e-7;
% % % % % % % % % % % Airl_max = 3.0e-7;
% % % % % % % % % % % Aorl_max = 3.0e-7;
% % % % % % % % % % % 
% % % % % % % % % % % % ---------- Sanitização ----------
% % % % % % % % % % % u_pwm = max(min(u_pwm, 100), -100);
% % % % % % % % % % % mcv   = double(mcv ~= 0);
% % % % % % % % % % % pfv   = double(pfv ~= 0);
% % % % % % % % % % % irl   = double(irl ~= 0);
% % % % % % % % % % % orl   = double(orl ~= 0);
% % % % % % % % % % % Psup  = max(Psup, Pret);
% % % % % % % % % % % Pw    = max(Pw,   Pret);
% % % % % % % % % % % x     = min(max(x, 0), x_max);
% % % % % % % % % % % 
% % % % % % % % % % % % ---------- Cinemática do LAC ----------
% % % % % % % % % % % v_cmd = K_drv * u_pwm;
% % % % % % % % % % % if (x <= 0 && v_cmd < 0)
% % % % % % % % % % %     x_dot = 0;
% % % % % % % % % % % elseif (x >= x_max && v_cmd > 0)
% % % % % % % % % % %     x_dot = 0;
% % % % % % % % % % % else
% % % % % % % % % % %     x_dot = v_cmd;
% % % % % % % % % % % end
% % % % % % % % % % % 
% % % % % % % % % % % % ---------- Vazões ----------
% % % % % % % % % % % Qlac_raw = A_p * x_dot;
% % % % % % % % % % % Qlac     = pfv * Qlac_raw;
% % % % % % % % % % % 
% % % % % % % % % % % dPmcv = max(Psup - Pret, 0);
% % % % % % % % % % % Qmcv  = mcv * Cv * Amcv_max * sqrt(2*dPmcv/rho);
% % % % % % % % % % % 
% % % % % % % % % % % dPin = max(Psup - Pw, 0);
% % % % % % % % % % % Qin  = irl * Cv * Airl_max * sqrt(2*dPin/rho);
% % % % % % % % % % % 
% % % % % % % % % % % dPout = max(Pw - Pret, 0);
% % % % % % % % % % % Qout  = orl * Cv * Aorl_max * sqrt(2*dPout/rho);
% % % % % % % % % % % 
% % % % % % % % % % % % ---------- Dinâmica das pressões (volume variável!) ----------
% % % % % % % % % % % %
% % % % % % % % % % % %  dP/dt = (beta / V(x)) × ΣQ
% % % % % % % % % % % %
% % % % % % % % % % % %  Vsup diminui com x → dP/dt AUMENTA com x → curva exponencial
% % % % % % % % % % % %
% % % % % % % % % % % Psup_dot = (beta / Vsup) * (Qlac - Qmcv - Qin);
% % % % % % % % % % % Pw_dot   = (beta / Vw)   * (Qin  - Qout);
% % % % % % % % % % % 
% % % % % % % % % % % end
% % % % % % % % % % % % function [Psup_dot, Pw_dot, x_dot, Qlac, Qmcv, Qin, Qout] = Bloco_Hidraulico_LAC( ...
% % % % % % % % % % % %     u_pwm, mcv, pfv, irl, orl, Psup, Pw, x)
% % % % % % % % % % % % % ---------------------------------------------------------------
% % % % % % % % % % % % % Bloco hidráulico LAC com MCV (malha aberta, 1 roda, sem CSV)
% % % % % % % % % % % % % ---------------------------------------------------------------
% % % % % % % % % % % % % Entradas:
% % % % % % % % % % % % %   u_pwm : comando do atuador [% PWM] (-100..+100)
% % % % % % % % % % % % %   mcv   : master cut valve, 0 = fechada, 1 = aberta (normal OPEN)
% % % % % % % % % % % % %   pfv   : pump feed valve,  0 = fechada, 1 = aberta (normal CLOSE)
% % % % % % % % % % % % %   irl   : inlet release valve, 0 = fechada, 1 = aberta (normal OPEN)
% % % % % % % % % % % % %   orl   : outlet release valve, 0 = fechada, 1 = aberta (normal CLOSE)
% % % % % % % % % % % % %   Psup  : pressão no manifold/suprimento [Pa]
% % % % % % % % % % % % %   Pw    : pressão na roda/caliper [Pa]
% % % % % % % % % % % % %   x     : posição do pistão do LAC [m]
% % % % % % % % % % % % %
% % % % % % % % % % % % % Saídas:
% % % % % % % % % % % % %   Psup_dot, Pw_dot  : derivadas de pressão [Pa/s]
% % % % % % % % % % % % %   x_dot             : velocidade do pistão [m/s]
% % % % % % % % % % % % %   Qlac, Qmcv, Qin, Qout : vazões [m^3/s]
% % % % % % % % % % % % % ---------------------------------------------------------------
% % % % % % % % % % % % 
% % % % % % % % % % % % % ---------- fluido / retorno ----------
% % % % % % % % % % % % % No início do seu Bloco Hidráulico
% % % % % % % % % % % % % beta = 1.5e9;          % VALOR ANTIGO (ideal, muito rígido)
% % % % % % % % % % % % beta = 0.08e9;         % VALOR NOVO (efetivo, ~20x mais complacente)
% % % % % % % % % % % % 
% % % % % % % % % % % % rho  = 850;            % kg/m^3
% % % % % % % % % % % % Pret = 1e5;            % Pa
% % % % % % % % % % % % 
% % % % % % % % % % % % % ---------- volumes efetivos ----------
% % % % % % % % % % % % Vsup = 6.0e-5;         % m^3
% % % % % % % % % % % % Vw   = 1.0e-5;         % m^3
% % % % % % % % % % % % 
% % % % % % % % % % % % % ---------- LAC ----------
% % % % % % % % % % % % D_mc  = 19.05e-3;
% % % % % % % % % % % % A_p   = pi*(D_mc/2)^2;              % ~2.85e-4 m^2
% % % % % % % % % % % % V_t   = 15.3e-6;                    % m^3
% % % % % % % % % % % % x_max = V_t / A_p;                  % curso hidráulico útil
% % % % % % % % % % % % 
% % % % % % % % % % % % % Driver fuso
% % % % % % % % % % % % mm_per_rev = 42.63/73;
% % % % % % % % % % % % m_per_rev  = mm_per_rev * 1e-3;
% % % % % % % % % % % % f_max_hz   = 46;
% % % % % % % % % % % % v_max_m_s  = f_max_hz * m_per_rev;
% % % % % % % % % % % % K_drv      = v_max_m_s / 100;       % (m/s) / %PWM
% % % % % % % % % % % % 
% % % % % % % % % % % % % ---------- válvulas ON/OFF (lei do orifício) ----------
% % % % % % % % % % % % Cv = 0.62;
% % % % % % % % % % % % 
% % % % % % % % % % % % % MCV — caminho mestre/reservatório (diâmetro maior, ~2 mm)
% % % % % % % % % % % % % Quando aberta, é praticamente sem resistência → área grande
% % % % % % % % % % % % Amcv_max = 3.0e-6;     % m^2 (~d=2.0 mm, baixa impedância)
% % % % % % % % % % % % 
% % % % % % % % % % % % % PFV — LAC → suprimento
% % % % % % % % % % % % Apfv_max = 3.0e-7;     % m^2 (~d=0.7 mm)
% % % % % % % % % % % % 
% % % % % % % % % % % % % IRL — suprimento → roda
% % % % % % % % % % % % Airl_max = 3.0e-7;     % m^2
% % % % % % % % % % % % 
% % % % % % % % % % % % % ORL — roda → retorno
% % % % % % % % % % % % Aorl_max = 3.0e-7;     % m^2
% % % % % % % % % % % % 
% % % % % % % % % % % % % Vazamentos
% % % % % % % % % % % % Kleak_sup = 0;
% % % % % % % % % % % % Kleak_w   = 0;
% % % % % % % % % % % % Kleak_lac = 0;
% % % % % % % % % % % % 
% % % % % % % % % % % % % ---------- sanitização ----------
% % % % % % % % % % % % u_pwm = max(min(u_pwm, 100), -100);
% % % % % % % % % % % % mcv   = double(mcv ~= 0);
% % % % % % % % % % % % pfv   = double(pfv ~= 0);
% % % % % % % % % % % % irl   = double(irl ~= 0);
% % % % % % % % % % % % orl   = double(orl ~= 0);
% % % % % % % % % % % % Psup  = max(Psup, Pret);
% % % % % % % % % % % % Pw    = max(Pw,   Pret);
% % % % % % % % % % % % x     = min(max(x, 0), x_max);
% % % % % % % % % % % % 
% % % % % % % % % % % % % ---------- cinemática do LAC ----------
% % % % % % % % % % % % v_cmd = K_drv * u_pwm;
% % % % % % % % % % % % if (x <= 0 && v_cmd < 0)
% % % % % % % % % % % %     x_dot = 0;
% % % % % % % % % % % % elseif (x >= x_max && v_cmd > 0)
% % % % % % % % % % % %     x_dot = 0;
% % % % % % % % % % % % else
% % % % % % % % % % % %     x_dot = v_cmd;
% % % % % % % % % % % % end
% % % % % % % % % % % % 
% % % % % % % % % % % % % ---------- vazões ----------
% % % % % % % % % % % % 
% % % % % % % % % % % % % LAC → suprimento (gated por PFV)
% % % % % % % % % % % % Qlac_raw = A_p * x_dot;
% % % % % % % % % % % % Qlac     = pfv * Qlac_raw - Kleak_lac*(Psup - Pret);
% % % % % % % % % % % % 
% % % % % % % % % % % % % MCV: suprimento ↔ reservatório (caminho de baixa impedância)
% % % % % % % % % % % % % Quando mcv=1 (aberta, estado normal): drena Psup para Pret
% % % % % % % % % % % % % Quando mcv=0 (fechada, energizada): isolada → LAC pode pressurizar
% % % % % % % % % % % % dPmcv = max(Psup - Pret, 0);
% % % % % % % % % % % % Qmcv  = mcv * Cv * Amcv_max * sqrt(2*dPmcv/rho);
% % % % % % % % % % % % 
% % % % % % % % % % % % % IRL: suprimento → roda
% % % % % % % % % % % % dPin = max(Psup - Pw, 0);
% % % % % % % % % % % % Qin  = irl * Cv * Airl_max * sqrt(2*dPin/rho);
% % % % % % % % % % % % 
% % % % % % % % % % % % % ORL: roda → retorno
% % % % % % % % % % % % dPout = max(Pw - Pret, 0);
% % % % % % % % % % % % Qout  = orl * Cv * Aorl_max * sqrt(2*dPout/rho);
% % % % % % % % % % % % 
% % % % % % % % % % % % % ---------- dinâmica das pressões ----------
% % % % % % % % % % % % %
% % % % % % % % % % % % %  Psup: entra Qlac, sai Qmcv, sai Qin
% % % % % % % % % % % % %  Pw:   entra Qin,  sai Qout
% % % % % % % % % % % % %
% % % % % % % % % % % % Psup_dot = (beta/Vsup) * (Qlac - Qmcv - Qin - Kleak_sup*(Psup - Pret));
% % % % % % % % % % % % Pw_dot   = (beta/Vw)   * (Qin  - Qout - Kleak_w*(Pw - Pret));
% % % % % % % % % % % % 
% % % % % % % % % % % % end
